simulink model "gm_HFMA_4B_1_5_9_13"  (R2026b)
settings: Solver=FixedStepDiscrete  StopTime=stopTime  FixedStep=1.953125e-06
PreLoadFcn:
  | load('a_luts.mat')
undefined symbols (not defined in the file or in its folder): Ts
libraries: simulink x202, simulink_need_slupdate x99, hdlsllib x91
(part 4 of 20)

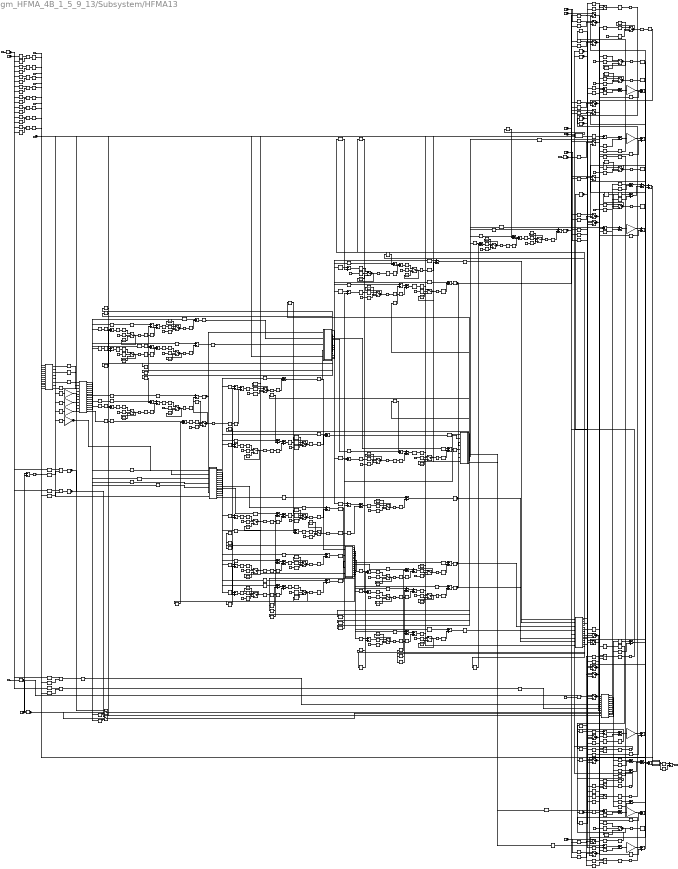
== system gm_HFMA_4B_1_5_9_13/Subsystem/HFMA13 ==
  Mic1 : Inport  OutDataTypeStr=fixdt(1, 20, 17)  PortDimensions=1  SampleTime=1.953125e-06
  Mic2 : Inport  Port=2  OutDataTypeStr=fixdt(1, 20, 17)  PortDimensions=1  SampleTime=1.953125e-06
  Mic3 : Inport  Port=3  OutDataTypeStr=fixdt(1, 20, 17)  PortDimensions=1  SampleTime=1.953125e-06
  Mic4 : Inport  Port=4  OutDataTypeStr=fixdt(1, 20, 17)  PortDimensions=1  SampleTime=1.953125e-06
  RESET : Inport  Port=5  OutDataTypeStr=boolean  PortDimensions=1  SampleTime=0.000125
  F0 Index : Inport  Port=6  OutDataTypeStr=fixdt(0, 18, 0)  PortDimensions=1  SampleTime=1.953125e-06
  IQ Counter : Inport  Port=7  OutDataTypeStr=uint8  PortDimensions=1  SampleTime=0.000125
  A Counter : Inport  Port=8  OutDataTypeStr=uint8  PortDimensions=1  SampleTime=0.000125
  sch_ctr_63 : Inport  Port=9  OutDataTypeStr=fixdt(0,6,0,'DataTypeOverride', 'Off')  PortDimensions=1  SampleTime=1.953125e-06
  Abs : Abs  SampleTime=1.953125e-06  OutDataTypeStr=fixdt(1, 18, 0)  SaturateOnIntegerOverflow=off
  Add : Sum  Inputs=+-  OutDataTypeStr=fixdt(1, 32, 29)  AccumDataTypeStr=fixdt(1, 33, 29)  SaturateOnIntegerOverflow=on  SampleTime=1.953125e-06
  Add1 : Sum  Inputs=+-  OutDataTypeStr=fixdt(1, 32, 29)  AccumDataTypeStr=fixdt(1, 33, 29)  SaturateOnIntegerOverflow=on  SampleTime=1.953125e-06
  Add{2..10} (9 alike) : Sum  OutDataTypeStr=fixdt(1, 32, 30)  AccumDataTypeStr=fixdt(1, 33, 30)  SaturateOnIntegerOverflow=on  SampleTime=1.953125e-06
  Add11 : Sum  OutDataTypeStr=fixdt(1, 32, 29)  AccumDataTypeStr=fixdt(1, 33, 29)  SaturateOnIntegerOverflow=on  SampleTime=1.953125e-06
  Add12 : Sum  OutDataTypeStr=fixdt(1, 32, 29)  AccumDataTypeStr=fixdt(1, 33, 29)  SaturateOnIntegerOverflow=on  SampleTime=1.953125e-06
  Add13 : Sum  Inputs=+-  OutDataTypeStr=fixdt(1, 32, 29)  AccumDataTypeStr=fixdt(1, 33, 29)  SaturateOnIntegerOverflow=on  SampleTime=1.953125e-06
  Add14 : Sum  OutDataTypeStr=fixdt(1, 32, 29)  AccumDataTypeStr=fixdt(1, 33, 29)  SaturateOnIntegerOverflow=on  SampleTime=1.953125e-06
  Add1_stage2 : Sum  OutDataTypeStr=fixdt(1, 34, 29)  AccumDataTypeStr=fixdt(1, 34, 29)  SaturateOnIntegerOverflow=on  SampleTime=1.953125e-06
  Add1_stage3 : Sum  OutDataTypeStr=fixdt(1, 32, 28)  AccumDataTypeStr=fixdt(1, 34, 29)  SaturateOnIntegerOverflow=on  SampleTime=1.953125e-06
  Add21 : Sum  OutDataTypeStr=fixdt(0, 40, 34)  AccumDataTypeStr=fixdt(0, 41, 34)  SaturateOnIntegerOverflow=on  SampleTime=1.953125e-06
  Add_stage2 : Sum  OutDataTypeStr=fixdt(1, 34, 29)  AccumDataTypeStr=fixdt(1, 34, 29)  SaturateOnIntegerOverflow=on  SampleTime=1.953125e-06
  Add_stage3 : Sum  OutDataTypeStr=fixdt(1, 32, 28)  AccumDataTypeStr=fixdt(1, 34, 29)  SaturateOnIntegerOverflow=on  SampleTime=1.953125e-06
  Compare : RelationalOperator  Operator===  OutDataTypeStr=boolean  SampleTime=1.953125e-06
  Constant : Constant  Value=90  OutDataTypeStr=fixdt(0, 18, 11)  SampleTime=1.953125e-06
  Constant1 : Constant  Value=180  OutDataTypeStr=uint8  SampleTime=1.953125e-06
  D1_{1..2,11..17,21..27} (16 alike) : RateTransition  OutPortSampleTimeOpt=Multiple of input port sample time  OutPortSampleTimeMultiple=64
  D1_1_absorbed{,1..7} (8 alike) : Delay  DelayLength=0
  D1_2_absorbed{,1..7} (8 alike) : Delay  DelayLength=0
  D2_{1..2,11..17,21..27} (16 alike) : RateTransition  OutPortSampleTimeOpt=Multiple of input port sample time  OutPortSampleTimeMultiple=64
  D2_1_absorbed{,1..7} (8 alike) : Delay  DelayLength=0
  D2_2_absorbed{,1..7} (8 alike) : Delay  DelayLength=0
  Delay1_bypass : Delay  DelayLength=1  InitialCondition=0  SampleTime=0.000125
  Delay1_bypass1 : RateTransition  OutPortSampleTimeOpt=Multiple of input port sample time  OutPortSampleTimeMultiple=64
  Delay1_lowered : RateTransition  OutPortSampleTimeOpt=Multiple of input port sample time  OutPortSampleTimeMultiple=64
  Delay1_lowered_absorbed : Delay  DelayLength=0
  Delay2_bypass : Delay  DelayLength=1  InitialCondition=0  SampleTime=0.000125
  Delay2_bypass1 : RateTransition  OutPortSampleTimeOpt=Multiple of input port sample time  OutPortSampleTimeMultiple=64
  Delay2_lowered : RateTransition  OutPortSampleTimeOpt=Multiple of input port sample time  OutPortSampleTimeMultiple=64
  Delay2_lowered_absorbed : Delay  DelayLength=0
  Delay3_bypass : Delay  DelayLength=1  InitialCondition=0  SampleTime=0.000125
  Delay3_bypass1 : RateTransition  OutPortSampleTimeOpt=Multiple of input port sample time  OutPortSampleTimeMultiple=64
  Delay3_lowered : RateTransition  OutPortSampleTimeOpt=Multiple of input port sample time  OutPortSampleTimeMultiple=64
  Delay3_lowered_absorbed : Delay  DelayLength=0
  Delay4_bypass : Delay  DelayLength=1  InitialCondition=0  SampleTime=0.000125
  Delay4_bypass1 : RateTransition  OutPortSampleTimeOpt=Multiple of input port sample time  OutPortSampleTimeMultiple=64
  Delay4_lowered : RateTransition  OutPortSampleTimeOpt=Multiple of input port sample time  OutPortSampleTimeMultiple=64
  Delay4_lowered_absorbed : Delay  DelayLength=0
  Delay5_bypass : Delay  DelayLength=1  InitialCondition=0  SampleTime=0.000125
  Delay5_bypass1 : RateTransition  OutPortSampleTimeOpt=Multiple of input port sample time  OutPortSampleTimeMultiple=64
  Delay5_lowered : RateTransition  OutPortSampleTimeOpt=Multiple of input port sample time  OutPortSampleTimeMultiple=64
  Delay5_lowered_absorbed : Delay  DelayLength=0
  Delay_Switch{,1..5} (6 alike) : Switch  Criteria=u2 ~= 0  OutDataTypeStr=fixdt(1, 32, 30)  SampleTime=1.953125e-06  SaturateOnIntegerOverflow=off  InputSameDT=off
  Delay_bypass : Delay  DelayLength=1  InitialCondition=0  SampleTime=0.000125
  Delay_bypass1 : RateTransition  OutPortSampleTimeOpt=Multiple of input port sample time  OutPortSampleTimeMultiple=64
  Delay_lowered{,1..6} (7 alike) : RateTransition  OutPortSampleTimeOpt=Multiple of input port sample time  OutPortSampleTimeMultiple=64
  Delay_lowered_absorbed{,1..6} (7 alike) : Delay  DelayLength=0
  Delay_toDelbypassMux{,1..5} (6 alike) : Switch  Criteria=u2 ~= 0  OutDataTypeStr=fixdt(1, 32, 30)  SampleTime=0.000125  SaturateOnIntegerOverflow=off  InputSameDT=off
  Direct Lookup Table (n-D) : LookupNDDirect  Table="reshape(fi([0.999969482421875;0.999969482421875;0.999969482421875;0.999969482421875;0.999969482421875;0.999969482421875;0.999969482421875;0.999969482421875;0.999969482421875;0.999969482421875;0.999969482421875;0.999969482421875;0.999969482421875;0.999969482421875;0.999969482421875;0.999969482421875;0.999969482421875;0.999969482421875;0.99993896484375;0.999908447265625;0.9998779296875;0.99981689453125;0.999755859375;0.99969482421875;0.9996337890625;0.99957275390625;0.999481201171875;0.9993896484375;0.999298095703125;0.999176025390625;0.99908447265625;0.99896240234375;0.99993896484375;0.9998779296875;0.999755859375;0.9996337890625;0.999481201171875;0.999298095703125;0.99908447265625;0.99884033203125;0.998565673828125;0.998260498046875;0.9979248046875;0.99755859375;0.997161865234375;0.99676513671875;0.996307373046875;0.995849609375;0.9998779296875;0.99969482421875;0.999481201171875;0.999176025390625;0.99884033203125;0.9984130859375;0.9979248046875;0.99737548828125;0.99676513671875;0.99609375;0.995330810546875;0.994537353515625;0.99365234375;0.992706298828125;0.99169921875;0.990631103515625;0.999755859375;0.999481201171875;0.99908447265625;0.998565673828125;0.9979248046875;0.9971923828125;0.996307373046875;0.995330810546875;0.994232177734375;0.9930419921875;0.991729736328125;0.99029541015625;0.988739013671875;0.987060546875;0.98529052734375;0.9833984375;0.9996337890625;0.999176025390625;0.998565673828125;0.99774169921875;0.99676513671875;0.99560546875;0.9942626953125;0.99273681640625;0.99102783203125;0.9891357421875;0.987091064453125;0.984832763671875;0.982421875;0.979827880859375;0.977081298828125;0.97412109375;0.999481201171875;0.99884033203125;0.9979248046875;0.99676513671875;0.995361328125;0.993682861328125;0.991729736328125;0.989532470703125;0.987091064453125;0.984375;0.9814453125;0.97821044921875;0.974761962890625;0.971038818359375;0.967071533203125;0.962860107421875;0.999298095703125;0.9984130859375;0.9971923828125;0.99560546875;0.993682861328125;0.99139404296875;0.98876953125;0.98577880859375;0.98248291015625;0.978790283203125;0.97479248046875;0.970428466796875;0.965728759765625;0.960693359375;0.955322265625;0.949615478515625;0.99908447265625;0.9979248046875;0.996337890625;0.9942626953125;0.99176025390625;0.988800048828125;0.9853515625;0.981475830078125;0.977142333984375;0.972381591796875;0.9671630859375;0.96148681640625;0.95538330078125;0.9488525390625;0.941864013671875;0.9344482421875;0.99884033203125;0.997406005859375;0.995361328125;0.992767333984375;0.989593505859375;0.98583984375;0.98150634765625;0.97662353515625;0.971160888671875;0.96514892578125;0.95855712890625;0.951446533203125;0.943756103515625;0.935516357421875;0.9267578125;0.917449951171875;0.998565673828125;0.996795654296875;0.994293212890625;0.9910888671875;0.9871826171875;0.9825439453125;0.97723388671875;0.971221923828125;0.964508056640625;0.957122802734375;0.94903564453125;0.940277099609375;0.93084716796875;0.920745849609375;0.910003662109375;0.898590087890625;0.998291015625;0.996124267578125;0.99310302734375;0.9892578125;0.984527587890625;0.97894287109375;0.9725341796875;0.965301513671875;0.95721435546875;0.94830322265625;0.938568115234375;0.92803955078125;0.916717529296875;0.904571533203125;0.89166259765625;0.87799072265625;0.997955322265625;0.995391845703125;0.9918212890625;0.98724365234375;0.98162841796875;0.97503662109375;0.967437744140625;0.958831787109375;0.949249267578125;0.938720703125;0.927215576171875;0.914764404296875;0.9013671875;0.887054443359375;0.871826171875;0.855712890625;0.99761962890625;0.994598388671875;0.99041748046875;0.98504638671875;0.978515625;0.970794677734375;0.9619140625;0.951873779296875;0.940673828125;0.928375244140625;0.91497802734375;0.90045166015625;0.884857177734375;0.86822509765625;0.85052490234375;0.831817626953125;0.997222900390625;0.9937744140625;0.988922119140625;0.98272705078125;0.97515869140625;0.96624755859375;0.95599365234375;0.94439697265625;0.9315185546875;0.917327880859375;0.901885986328125;0.885162353515625 ...(+21044 chars)), [16  91])"  SampleTime=1.953125e-06  TableDataTypeStr=fixdt(1,18,16)
  Direct Lookup Table (n-D)1 : LookupNDDirect  Table="reshape(fi([0;0;0;0;0;0;0;0;0;0;0;0;0;0;0;0;-0.00537109375;-0.008056640625;-0.0107421875;-0.013427734375;-0.01611328125;-0.018798828125;-0.021484375;-0.024169921875;-0.02685546875;-0.029541015625;-0.0322265625;-0.034912109375;-0.03759765625;-0.040283203125;-0.04296875;-0.045623779296875;-0.0107421875;-0.01611328125;-0.021484375;-0.02685546875;-0.0322265625;-0.037567138671875;-0.042938232421875;-0.048309326171875;-0.053680419921875;-0.059051513671875;-0.06439208984375;-0.06976318359375;-0.075103759765625;-0.080474853515625;-0.0858154296875;-0.091156005859375;-0.01611328125;-0.024169921875;-0.032196044921875;-0.040252685546875;-0.048309326171875;-0.05633544921875;-0.06439208984375;-0.072418212890625;-0.0804443359375;-0.088470458984375;-0.09649658203125;-0.1044921875;-0.112518310546875;-0.120513916015625;-0.12847900390625;-0.136474609375;-0.021453857421875;-0.032196044921875;-0.04290771484375;-0.05364990234375;-0.064361572265625;-0.0750732421875;-0.08575439453125;-0.096466064453125;-0.10711669921875;-0.1177978515625;-0.128448486328125;-0.13909912109375;-0.14971923828125;-0.160308837890625;-0.1708984375;-0.18145751953125;-0.026824951171875;-0.04022216796875;-0.053619384765625;-0.0670166015625;-0.08038330078125;-0.09375;-0.107086181640625;-0.120391845703125;-0.133697509765625;-0.14697265625;-0.160247802734375;-0.1734619140625;-0.1866455078125;-0.199798583984375;-0.212921142578125;-0.22601318359375;-0.03216552734375;-0.048248291015625;-0.064300537109375;-0.080322265625;-0.096343994140625;-0.11236572265625;-0.128326416015625;-0.144256591796875;-0.16015625;-0.175994873046875;-0.191802978515625;-0.20758056640625;-0.2232666015625;-0.238922119140625;-0.2545166015625;-0.270050048828125;-0.037506103515625;-0.05621337890625;-0.074951171875;-0.0936279296875;-0.112274169921875;-0.130889892578125;-0.149444580078125;-0.16796875;-0.186431884765625;-0.204803466796875;-0.22314453125;-0.241363525390625;-0.259521484375;-0.277587890625;-0.295562744140625;-0.31341552734375;-0.042816162109375;-0.064208984375;-0.085540771484375;-0.10687255859375;-0.128143310546875;-0.14935302734375;-0.17047119140625;-0.191558837890625;-0.2125244140625;-0.2333984375;-0.254150390625;-0.274810791015625;-0.29534912109375;-0.31573486328125;-0.335968017578125;-0.3560791015625;-0.048126220703125;-0.0721435546875;-0.09613037109375;-0.12005615234375;-0.1439208984375;-0.167694091796875;-0.191375732421875;-0.214935302734375;-0.2384033203125;-0.261688232421875;-0.28485107421875;-0.307830810546875;-0.330657958984375;-0.353271484375;-0.375701904296875;-0.39788818359375;-0.05340576171875;-0.080078125;-0.106689453125;-0.133209228515625;-0.159637451171875;-0.185943603515625;-0.212127685546875;-0.2381591796875;-0.2640380859375;-0.289703369140625;-0.315185546875;-0.340423583984375;-0.36541748046875;-0.390167236328125;-0.41461181640625;-0.43878173828125;-0.058685302734375;-0.087982177734375;-0.1171875;-0.146270751953125;-0.175262451171875;-0.204071044921875;-0.23272705078125;-0.26116943359375;-0.289398193359375;-0.3173828125;-0.3450927734375;-0.37249755859375;-0.399566650390625;-0.426300048828125;-0.452667236328125;-0.478668212890625;-0.063934326171875;-0.0958251953125;-0.12762451171875;-0.159271240234375;-0.190765380859375;-0.222076416015625;-0.253143310546875;-0.283966064453125;-0.314483642578125;-0.344696044921875;-0.374542236328125;-0.404022216796875;-0.433074951171875;-0.461669921875;-0.48980712890625;-0.5174560546875;-0.069183349609375;-0.103668212890625;-0.13800048828125;-0.172210693359375;-0.206207275390625;-0.23992919921875;-0.27337646484375;-0.3065185546875;-0.339263916015625;-0.371612548828125;-0.403533935546875;-0.4349365234375;-0.465850830078125;-0.496185302734375;-0.52593994140625;-0.5550537109375;-0.074371337890625;-0.1114501953125;-0.148345947265625;-0.18505859375;-0.22149658203125;-0.25762939453125;-0.293426513671875;-0.32879638671875;-0.36370849609375;-0.39813232421875;-0.4320068359375;-0.46527099609375;-0.497894287109375;-0.529815673828125;-0.561004638671875;-0.5914306640625 ...(+21853 chars)), [16  91])"  SampleTime=1.953125e-06  TableDataTypeStr=fixdt(1,18,16)
  Direct Lookup Table (n-D)2 : LookupNDDirect  Table="reshape(fi([0.999969482421875;0.999969482421875;0.999969482421875;0.999969482421875;0.999969482421875;0.999969482421875;0.999969482421875;0.999969482421875;0.999969482421875;0.999969482421875;0.999969482421875;0.999969482421875;0.999969482421875;0.999969482421875;0.999969482421875;0.999969482421875;0.99993896484375;0.9998779296875;0.999755859375;0.9996337890625;0.999481201171875;0.999298095703125;0.99908447265625;0.99884033203125;0.998565673828125;0.998260498046875;0.9979248046875;0.99755859375;0.997161865234375;0.99676513671875;0.996307373046875;0.995849609375;0.999755859375;0.999481201171875;0.99908447265625;0.998565673828125;0.9979248046875;0.997161865234375;0.996307373046875;0.995330810546875;0.994232177734375;0.9930419921875;0.99169921875;0.990264892578125;0.98870849609375;0.987060546875;0.985260009765625;0.983367919921875;0.999481201171875;0.99884033203125;0.9979248046875;0.99676513671875;0.995330810546875;0.99365234375;0.99169921875;0.989501953125;0.987060546875;0.984344482421875;0.98138427734375;0.9781494140625;0.97467041015625;0.970947265625;0.96697998046875;0.962738037109375;0.99908447265625;0.9979248046875;0.996307373046875;0.994232177734375;0.991729736328125;0.988739013671875;0.98529052734375;0.98138427734375;0.97705078125;0.972259521484375;0.967010498046875;0.9613037109375;0.955169677734375;0.9486083984375;0.94158935546875;0.93414306640625;0.998565673828125;0.99676513671875;0.9942626953125;0.99102783203125;0.987091064453125;0.982421875;0.977081298828125;0.97100830078125;0.9642333984375;0.956787109375;0.948638916015625;0.9398193359375;0.930328369140625;0.920166015625;0.909332275390625;0.8978271484375;0.9979248046875;0.995361328125;0.991729736328125;0.987091064453125;0.9814453125;0.974761962890625;0.967071533203125;0.9583740234375;0.948699951171875;0.93804931640625;0.926422119140625;0.913818359375;0.900299072265625;0.885833740234375;0.870452880859375;0.854156494140625;0.9971923828125;0.993682861328125;0.98876953125;0.98248291015625;0.97479248046875;0.965728759765625;0.955322265625;0.943572998046875;0.93048095703125;0.916107177734375;0.900421142578125;0.88348388671875;0.86529541015625;0.84588623046875;0.825286865234375;0.80352783203125;0.996337890625;0.99176025390625;0.9853515625;0.977142333984375;0.9671630859375;0.95538330078125;0.941864013671875;0.9266357421875;0.90966796875;0.89105224609375;0.87078857421875;0.848968505859375;0.8255615234375;0.800628662109375;0.77423095703125;0.746429443359375;0.995361328125;0.989593505859375;0.98150634765625;0.971160888671875;0.95855712890625;0.943756103515625;0.9267578125;0.9075927734375;0.886322021484375;0.863037109375;0.83770751953125;0.810455322265625;0.781341552734375;0.750396728515625;0.71771240234375;0.683380126953125;0.994293212890625;0.9871826171875;0.97723388671875;0.964508056640625;0.94903564453125;0.93084716796875;0.910003662109375;0.886566162109375;0.860565185546875;0.8321533203125;0.80133056640625;0.768218994140625;0.732940673828125;0.695556640625;0.65618896484375;0.614959716796875;0.99310302734375;0.984527587890625;0.9725341796875;0.95721435546875;0.938568115234375;0.916717529296875;0.89166259765625;0.863555908203125;0.832489013671875;0.798553466796875;0.7618408203125;0.722503662109375;0.680694580078125;0.63653564453125;0.59014892578125;0.541778564453125;0.9918212890625;0.98162841796875;0.967437744140625;0.949249267578125;0.927215576171875;0.9013671875;0.871826171875;0.838714599609375;0.80218505859375;0.762359619140625;0.71942138671875;0.673553466796875;0.624908447265625;0.573699951171875;0.520172119140625;0.464508056640625;0.99041748046875;0.978515625;0.9619140625;0.940673828125;0.91497802734375;0.884857177734375;0.85052490234375;0.812103271484375;0.769805908203125;0.723785400390625;0.67431640625;0.62164306640625;0.565948486328125;0.507568359375;0.44677734375;0.383819580078125;0.988922119140625;0.97515869140625;0.95599365234375;0.9315185546875;0.901885986328125;0.86724853515625;0.82781982421875;0.783782958984375;0.73541259765625;0.6829833984375;0.62677001953125 ...(+21447 chars)), [16  91])"  SampleTime=1.953125e-06  TableDataTypeStr=fixdt(1,18,16)
  Direct Lookup Table (n-D)3 : LookupNDDirect  Table="reshape(fi([0;0;0;0;0;0;0;0;0;0;0;0;0;0;0;0;-0.0107421875;-0.01611328125;-0.021484375;-0.02685546875;-0.0322265625;-0.03759765625;-0.04296875;-0.048309326171875;-0.053680419921875;-0.059051513671875;-0.06439208984375;-0.06976318359375;-0.07513427734375;-0.080474853515625;-0.0858154296875;-0.0911865234375;-0.021484375;-0.0322265625;-0.042938232421875;-0.053680419921875;-0.06439208984375;-0.075103759765625;-0.0858154296875;-0.09649658203125;-0.107208251953125;-0.11785888671875;-0.1285400390625;-0.13916015625;-0.149810791015625;-0.160400390625;-0.170989990234375;-0.18157958984375;-0.032196044921875;-0.048309326171875;-0.06439208984375;-0.0804443359375;-0.09649658203125;-0.112518310546875;-0.12847900390625;-0.144439697265625;-0.160369873046875;-0.176239013671875;-0.19207763671875;-0.207855224609375;-0.22357177734375;-0.2392578125;-0.254852294921875;-0.2703857421875;-0.04290771484375;-0.064361572265625;-0.08575439453125;-0.10711669921875;-0.128448486328125;-0.14971923828125;-0.1708984375;-0.1920166015625;-0.213043212890625;-0.23394775390625;-0.2547607421875;-0.275482177734375;-0.296051025390625;-0.31646728515625;-0.336761474609375;-0.356903076171875;-0.053619384765625;-0.08038330078125;-0.107086181640625;-0.133697509765625;-0.160247802734375;-0.1866455078125;-0.212921142578125;-0.23907470703125;-0.2650146484375;-0.290771484375;-0.31634521484375;-0.3416748046875;-0.36676025390625;-0.391571044921875;-0.416107177734375;-0.440338134765625;-0.064300537109375;-0.096343994140625;-0.128326416015625;-0.16015625;-0.191802978515625;-0.2232666015625;-0.2545166015625;-0.285491943359375;-0.316162109375;-0.346527099609375;-0.376495361328125;-0.406097412109375;-0.435302734375;-0.464019775390625;-0.492279052734375;-0.52001953125;-0.074951171875;-0.112274169921875;-0.149444580078125;-0.186431884765625;-0.22314453125;-0.259521484375;-0.295562744140625;-0.3311767578125;-0.3663330078125;-0.40093994140625;-0.435028076171875;-0.468475341796875;-0.50128173828125;-0.533355712890625;-0.564697265625;-0.595245361328125;-0.085540771484375;-0.128143310546875;-0.17047119140625;-0.2125244140625;-0.254150390625;-0.29534912109375;-0.335968017578125;-0.376007080078125;-0.415313720703125;-0.453887939453125;-0.49163818359375;-0.528472900390625;-0.5643310546875;-0.599151611328125;-0.632904052734375;-0.66546630859375;-0.09613037109375;-0.1439208984375;-0.191375732421875;-0.2384033203125;-0.28485107421875;-0.330657958984375;-0.375701904296875;-0.41986083984375;-0.463043212890625;-0.505157470703125;-0.546112060546875;-0.585784912109375;-0.624114990234375;-0.660980224609375;-0.696319580078125;-0.730072021484375;-0.106689453125;-0.159637451171875;-0.212127685546875;-0.2640380859375;-0.315185546875;-0.36541748046875;-0.41461181640625;-0.462615966796875;-0.50933837890625;-0.5545654296875;-0.59820556640625;-0.640167236328125;-0.6802978515625;-0.718475341796875;-0.754608154296875;-0.78857421875;-0.1171875;-0.175262451171875;-0.23272705078125;-0.289398193359375;-0.3450927734375;-0.399566650390625;-0.452667236328125;-0.504241943359375;-0.554046630859375;-0.6019287109375;-0.64776611328125;-0.691375732421875;-0.732574462890625;-0.771270751953125;-0.807281494140625;-0.84051513671875;-0.12762451171875;-0.190765380859375;-0.253143310546875;-0.314483642578125;-0.374542236328125;-0.433074951171875;-0.48980712890625;-0.5445556640625;-0.597076416015625;-0.64715576171875;-0.694549560546875;-0.7391357421875;-0.78070068359375;-0.819061279296875;-0.85406494140625;-0.885589599609375;-0.13800048828125;-0.206207275390625;-0.27337646484375;-0.339263916015625;-0.403533935546875;-0.465850830078125;-0.52593994140625;-0.583526611328125;-0.6383056640625;-0.69000244140625;-0.738433837890625;-0.783294677734375;-0.824432373046875;-0.861602783203125;-0.8946533203125;-0.92340087890625;-0.148345947265625;-0.22149658203125;-0.293426513671875;-0.36370849609375;-0.4320068359375;-0.497894287109375;-0.561004638671875;-0.62103271484375;-0.6776123046875;-0.730438232421875;-0.779205322265625;-0.82366943359375 ...(+21735 chars)), [16  91])"  SampleTime=1.953125e-06  TableDataTypeStr=fixdt(1,18,16)
  Gain{,1..5} (6 alike) : Gain  Gain="fi(0,1,32,40,\"hex\",\"40000000\")"  ParamDataTypeStr=fixdt(1, 32, 40)  OutDataTypeStr=fixdt(1, 32, 30)  SaturateOnIntegerOverflow=on  SampleTime=1.953125e-06
  Gain{11..14} (4 alike) : Gain  Gain="fi(0,0,18,16,\"hex\",\"20000\")"  ParamDataTypeStr=fixdt(0, 18, 16)  OutDataTypeStr=fixdt(1, 18, 14)  SaturateOnIntegerOverflow=on  SampleTime=1.953125e-06
  Gain1_out_dtc : DataTypeConversion  OutDataTypeStr=fixdt(0, 18, 17)  SampleTime=1.953125e-06  RndMeth=Floor
  Gain_out_dtc : DataTypeConversion  OutDataTypeStr=fixdt(1, 18, 16)  SampleTime=1.953125e-06  RndMeth=Floor
  Gain_out_dtc{1..4} (4 alike) : DataTypeConversion  OutDataTypeStr=fixdt(1, 18, 14)  SampleTime=1.953125e-06  RndMeth=Floor
  IdxConv{,2..10,14..15,21..24} (16 alike) : DataTypeConversion  OutDataTypeStr=uint8  SampleTime=1.953125e-06  RndMeth=Floor
  IdxConv{1,11..13,31..34} (8 alike) : DataTypeConversion  OutDataTypeStr=fixdt('uint8')
  Initial_Val{,1..5} (6 alike) : Constant  Value=0  OutDataTypeStr=fixdt(1, 32, 30)  SampleTime=1.953125e-06
  Minus{,1..5} (6 alike) : Sum  Inputs=+-  OutDataTypeStr=fixdt(1, 32, 30)  AccumDataTypeStr=fixdt(1, 33, 30)  SaturateOnIntegerOverflow=on  SampleTime=1.953125e-06
  PipelineRegister{,1..11} (12 alike) : Delay  DelayLength=1  InitialCondition=0  SampleTime=1.953125e-06
  Product1_out_dtc : DataTypeConversion  OutDataTypeStr=fixdt(1, 32, 29)  SampleTime=1.953125e-06  RndMeth=Floor
  Product1_out_dtc1 : DataTypeConversion  OutDataTypeStr=fixdt(1, 32, 29)  SampleTime=1.953125e-06  RndMeth=Floor
  Product1_out_dtc{4,6..8,10..11} (6 alike) : DataTypeConversion  OutDataTypeStr=fixdt(1, 32, 30)  SampleTime=1.953125e-06  RndMeth=Floor
  Product1_out_dtc{3,5,9,12} (4 alike) : DataTypeConversion  OutDataTypeStr=fixdt(1, 18, 15)  SampleTime=1.953125e-06  RndMeth=Floor
  Product1_out_dtc13 : DataTypeConversion  OutDataTypeStr=fixdt(0, 40, 34)  SampleTime=1.953125e-06  RndMeth=Floor
  Product1_out_dtc2 : DataTypeConversion  OutDataTypeStr=fixdt(1, 32, 29)  SampleTime=1.953125e-06  RndMeth=Floor
  Product2_out_dtc : DataTypeConversion  OutDataTypeStr=fixdt(1, 32, 29)  SampleTime=1.953125e-06  RndMeth=Floor
  Product2_out_dtc1 : DataTypeConversion  OutDataTypeStr=fixdt(1, 32, 29)  SampleTime=1.953125e-06  RndMeth=Floor
  Product2_out_dtc2 : DataTypeConversion  OutDataTypeStr=fixdt(1, 32, 29)  SampleTime=1.953125e-06  RndMeth=Floor
  Product3_out_dtc : DataTypeConversion  OutDataTypeStr=fixdt(1, 32, 29)  SampleTime=1.953125e-06  RndMeth=Floor
  Product3_out_dtc1 : DataTypeConversion  OutDataTypeStr=fixdt(1, 32, 29)  SampleTime=1.953125e-06  RndMeth=Floor
  Product3_out_dtc2 : DataTypeConversion  OutDataTypeStr=fixdt(1, 32, 29)  SampleTime=1.953125e-06  RndMeth=Floor
  Product_out_dtc : DataTypeConversion  OutDataTypeStr=fixdt(1, 32, 29)  SampleTime=1.953125e-06  RndMeth=Floor
  Product_out_dtc1 : DataTypeConversion  OutDataTypeStr=fixdt(1, 32, 29)  SampleTime=1.953125e-06  RndMeth=Floor
  Product_out_dtc{3..4,6,8,10..11} (6 alike) : DataTypeConversion  OutDataTypeStr=fixdt(1, 32, 30)  SampleTime=1.953125e-06  RndMeth=Floor
  Product_out_dtc12 : DataTypeConversion  OutDataTypeStr=fixdt(1, 32, 29)  SampleTime=1.953125e-06  RndMeth=Floor
  Product_out_dtc13 : DataTypeConversion  OutDataTypeStr=fixdt(0, 40, 34)  SampleTime=1.953125e-06  RndMeth=Floor
  Product_out_dtc{2,5,7,9} (4 alike) : DataTypeConversion  OutDataTypeStr=fixdt(1, 18, 15)  SampleTime=1.953125e-06  RndMeth=Floor
  Q_{1..2,11..17,21..27} (16 alike) : DataTypeConversion  OutDataTypeStr=fixdt(1, 18, 16)  SampleTime=1.953125e-06  RndMeth=Floor
  Relational Operator : RelationalOperator  OutDataTypeStr=boolean  SampleTime=1.953125e-06  InputSameDT=off
  S0_{1..2,11..17,21..27} (16 alike) : Sum  OutDataTypeStr=fixdt(1, 40, 30)  AccumDataTypeStr=fixdt(1, 41, 30)  SaturateOnIntegerOverflow=on  SampleTime=1.953125e-06
  S1_1_out1bypassMux{,1..7} (8 alike) : Switch  Criteria=u2 ~= 0  OutDataTypeStr=fixdt(1, 40, 30)  SampleTime=0.000125  SaturateOnIntegerOverflow=off  InputSameDT=off
  S1_1_stage{2,21..27} (8 alike) : Sum  OutDataTypeStr=fixdt(1, 42, 30)  AccumDataTypeStr=fixdt(1, 42, 30)  SaturateOnIntegerOverflow=on  SampleTime=1.953125e-06
  S1_1_stage{3,31..37} (8 alike) : Sum  OutDataTypeStr=fixdt(1, 40, 30)  AccumDataTypeStr=fixdt(1, 42, 30)  SaturateOnIntegerOverflow=on  SampleTime=1.953125e-06
  S1_2_out1bypassMux{,1..7} (8 alike) : Switch  Criteria=u2 ~= 0  OutDataTypeStr=fixdt(1, 40, 30)  SampleTime=0.000125  SaturateOnIntegerOverflow=off  InputSameDT=off
  S1_2_stage{2,21..27} (8 alike) : Sum  OutDataTypeStr=fixdt(1, 42, 30)  AccumDataTypeStr=fixdt(1, 42, 30)  SaturateOnIntegerOverflow=on  SampleTime=1.953125e-06
  S1_2_stage{3,31..37} (8 alike) : Sum  OutDataTypeStr=fixdt(1, 40, 30)  AccumDataTypeStr=fixdt(1, 42, 30)  SaturateOnIntegerOverflow=on  SampleTime=1.953125e-06
  S2_{1..2,11..17,21..27} (16 alike) : Sum  OutDataTypeStr=fixdt(1, 40, 30)  AccumDataTypeStr=fixdt(1, 41, 30)  SaturateOnIntegerOverflow=on  SampleTime=1.953125e-06
  S2_1_out1bypassMux{,1..7} (8 alike) : Switch  Criteria=u2 ~= 0  OutDataTypeStr=fixdt(1, 40, 30)  SampleTime=0.000125  SaturateOnIntegerOverflow=off  InputSameDT=off
  S2_2_out1bypassMux{,1..7} (8 alike) : Switch  Criteria=u2 ~= 0  OutDataTypeStr=fixdt(1, 40, 30)  SampleTime=0.000125  SaturateOnIntegerOverflow=off  InputSameDT=off
  Subtract : Sum  Inputs=+-  OutDataTypeStr=fixdt(1, 18, 0)  AccumDataTypeStr=fixdt(1, 20, 11)  SaturateOnIntegerOverflow=on  SampleTime=1.953125e-06
  Subtract1 : Sum  Inputs=+-  OutDataTypeStr=fixdt(1, 32, 30)  AccumDataTypeStr=fixdt(1, 33, 30)  SaturateOnIntegerOverflow=on  SampleTime=1.953125e-06
  Subtract2 : Sum  Inputs=+-  OutDataTypeStr=fixdt(1, 32, 30)  AccumDataTypeStr=fixdt(1, 33, 30)  SaturateOnIntegerOverflow=on  SampleTime=1.953125e-06
  Subtract3 : Sum  Inputs=+-  OutDataTypeStr=fixdt(1, 32, 30)  AccumDataTypeStr=fixdt(1, 33, 30)  SaturateOnIntegerOverflow=on  SampleTime=1.953125e-06
  Switch : Switch  Criteria=u2 ~= 0  Threshold="fi(0,0,1,0,\"hex\",\"0\")"  OutDataTypeStr=fixdt(1, 18, 16)  SampleTime=1.953125e-06  SaturateOnIntegerOverflow=off  InputSameDT=off
  Switch1 : Switch  Criteria=u2 ~= 0  Threshold="fi(0,0,1,0,\"hex\",\"0\")"  OutDataTypeStr=fixdt(1, 18, 16)  SampleTime=1.953125e-06  SaturateOnIntegerOverflow=off  InputSameDT=off
  b0_1_out_dtc{,1..7} (8 alike) : DataTypeConversion  OutDataTypeStr=fixdt(1, 40, 30)  SampleTime=1.953125e-06  RndMeth=Floor
  b0_2_out_dtc{,1..7} (8 alike) : DataTypeConversion  OutDataTypeStr=fixdt(1, 40, 30)  SampleTime=1.953125e-06  RndMeth=Floor
  b1_1_out_dtc{,1..7} (8 alike) : DataTypeConversion  OutDataTypeStr=fixdt(1, 40, 30)  SampleTime=1.953125e-06  RndMeth=Floor
  b1_2_out_dtc{,1..7} (8 alike) : DataTypeConversion  OutDataTypeStr=fixdt(1, 40, 30)  SampleTime=1.953125e-06  RndMeth=Floor
  b2_1_out_dtc{,1..7} (8 alike) : DataTypeConversion  OutDataTypeStr=fixdt(1, 40, 30)  SampleTime=1.953125e-06  RndMeth=Floor
  b2_2_out_dtc{,1..7} (8 alike) : DataTypeConversion  OutDataTypeStr=fixdt(1, 40, 30)  SampleTime=1.953125e-06  RndMeth=Floor
  bypass_out{,1..5} (6 alike) : Switch  Criteria=u2 ~= 0  OutDataTypeStr=fixdt(1, 32, 30)  SampleTime=1.953125e-06  SaturateOnIntegerOverflow=off  InputSameDT=off
  cosLUT{,1..3} (4 alike) : LookupNDDirect  Table="reshape([1;1;1;1;1;1;1;1;1;1;1;1;1;1;1;1;0.95105651629515353;0.8910065241883679;0.80901699437494745;0.70710678118654757;0.58778525229247314;0.45399049973954686;0.30901699437494745;0.15643446504023092;6.123233995736766e-17;-0.15643446504023081;-0.30901699437494734;-0.45399049973954675;-0.58778525229247303;-0.70710678118654746;-0.80901699437494734;-0.89100652418836779;0.80901699437494745;0.58778525229247314;0.30901699437494745;6.123233995736766e-17;-0.30901699437494734;-0.58778525229247303;-0.80901699437494734;-0.95105651629515353;-1;-0.95105651629515364;-0.80901699437494745;-0.58778525229247325;-0.30901699437494756;-1.8369701987210297e-16;0.30901699437494723;0.58778525229247292;0.58778525229247314;0.15643446504023092;-0.30901699437494734;-0.70710678118654746;-0.95105651629515353;-0.98768834059513777;-0.80901699437494745;-0.45399049973954692;-1.8369701987210297e-16;0.45399049973954664;0.80901699437494734;0.98768834059513755;0.95105651629515398;0.70710678118654835;0.30901699437494773;-0.15643446504022968;0.30901699437494745;-0.30901699437494734;-0.80901699437494734;-1;-0.80901699437494745;-0.30901699437494756;0.30901699437494723;0.80901699437494734;1;0.80901699437494756;0.30901699437494773;-0.30901699437494712;-0.80901699437494723;-1;-0.80901699437494767;-0.30901699437494784;-1.6081226496766366e-16;-0.70710678118654746;-1;-0.70710678118654791;-1.8369701987210297e-16;0.70710678118654735;1;0.70710678118654835;1.1943401194869635e-15;-0.70710678118654791;-1;-0.70710678118654846;-4.2862637970157361e-16;0.70710678118654779;1;0.70710678118654857;-0.30901699437494734;-0.95105651629515353;-0.80901699437494745;-1.8369701987210297e-16;0.80901699437494734;0.95105651629515398;0.30901699437494773;-0.58778525229247292;-1;-0.58778525229247347;0.30901699437494701;0.95105651629515287;0.80901699437494878;2.3274478990165594e-15;-0.80901699437494712;-0.95105651629515431;-0.58778525229247336;-0.98768834059513777;-0.30901699437494673;0.70710678118654735;0.95105651629515364;0.15643446504023203;-0.80901699437494823;-0.89100652418836768;-4.2862637970157361e-16;0.89100652418836801;0.80901699437494778;-0.15643446504022945;-0.95105651629515287;-0.70710678118654735;0.30901699437495017;0.98768834059513744;-0.80901699437494734;-0.80901699437494745;0.30901699437494723;1;0.30901699437494773;-0.80901699437494723;-0.80901699437494767;0.30901699437494701;1;0.30901699437494795;-0.80901699437494712;-0.80901699437494778;0.30901699437494679;1;0.30901699437494817;-0.8090169943749469;-0.95105651629515353;-0.45399049973954692;0.80901699437494734;0.70710678118654835;-0.58778525229247292;-0.89100652418836845;0.30901699437494701;0.98768834059513799;2.3274478990165594e-15;-0.98768834059513777;-0.30901699437494806;0.89100652418836634;0.58778525229247514;-0.70710678118654635;-0.8090169943749479;0.45399049973954675;-1;-1.8369701987210297e-16;1;1.1943401194869635e-15;-1;-4.2862637970157361e-16;1;2.3274478990165594e-15;-1;1.1028010998692062e-15;1;2.5723772588460301e-15;-1;8.5787174003973557e-16;1;2.8173066186755008e-15;-0.95105651629515364;0.45399049973954581;0.80901699437494756;-0.70710678118654668;-0.58778525229247491;0.89100652418836723;0.30901699437494795;-0.98768834059513777;-2.4499125789312946e-15;0.98768834059513766;-0.30901699437494329;-0.89100652418836868;0.58778525229247092;0.70710678118654757;-0.80901699437494679;-0.45399049973955174;-0.80901699437494745;0.80901699437494734;0.30901699437494773;-1;0.30901699437494701;0.80901699437494878;-0.80901699437494712;-0.30901699437494806;1;-0.30901699437494667;-0.8090169943749479;0.80901699437494479;0.30901699437495178;-1;0.30901699437494629;0.80901699437495023;-0.58778525229247325;0.98768834059513766;-0.30901699437494712;-0.70710678118654846;0.95105651629515342;-0.15643446504022945;-0.80901699437494778;0.8910065241883679;2.5723772588460301e-15;-0.89100652418836701;0.8090169943749469;0.15643446504023453;-0.95105651629515442;0.70710678118654602;0.30901699437494862;-0.98768834059513833;-0.30901699437494673;0.95105651629515364 ...(+7561 chars)])"  SampleTime=1.953125e-06  TableDataTypeStr=fixdt(1,18,16)
  crp_out_delay{,1..23} (24 alike) : Delay  DelayLength=1  InitialCondition=0  SampleTime=1.953125e-06
  crp_temp_shared : Subsystem
  crp_temp_shared1 : Subsystem
  crp_temp_shared2 : Subsystem
  crp_temp_shared3 : Subsystem
  crp_temp_shared4 : Subsystem
  crp_temp_shared5 : Subsystem
  crp_temp_shared6 : Subsystem
  crp_temp_shared7 : Subsystem
  crp_temp_shared8 : Subsystem
  crp_temp_shared9 : Subsystem
  delayMatch{,1,3..4,6..7,9..10,12..15,17..18,21..24,27..28,31..34,37..40,43..44,48..49,52..53,56..57,60..61,64..65} (40 alike) : Delay  DelayLength=1  InitialCondition=0  SampleTime=1.953125e-06
  delayMatch{66..103} (38 alike) : Delay  DelayLength=1  InitialCondition=0  SampleTime=0.000125
  delayMatch{2,5,8,11,16,19} (6 alike) : Delay  DelayLength=65  InitialCondition=0  SampleTime=1.953125e-06
  delayMatch{20,25..26,29..30,35..36} (7 alike) : Delay  DelayLength=25  InitialCondition=0  SampleTime=1.953125e-06
  delayMatch{41..42,46..47,50..51,54..55,58..59,62..63} (12 alike) : Delay  DelayLength=64  InitialCondition=0  SampleTime=1.953125e-06
  delayMatch45 : Delay  DelayLength=9  InitialCondition=0  SampleTime=1.953125e-06
  in0_repeat : RateTransition  Integrity=off  Deterministic=off  OutPortSampleTimeOpt=Multiple of input port sample time  OutPortSampleTimeMultiple=1/64
  in10_repeat : RateTransition  Integrity=off  Deterministic=off  OutPortSampleTimeOpt=Multiple of input port sample time  OutPortSampleTimeMultiple=1/64
  in11_repeat : RateTransition  Integrity=off  Deterministic=off  OutPortSampleTimeOpt=Multiple of input port sample time  OutPortSampleTimeMultiple=1/64
  in12_repeat : RateTransition  Integrity=off  Deterministic=off  OutPortSampleTimeOpt=Multiple of input port sample time  OutPortSampleTimeMultiple=1/64
  in13_repeat : RateTransition  Integrity=off  Deterministic=off  OutPortSampleTimeOpt=Multiple of input port sample time  OutPortSampleTimeMultiple=1/64
  in14_repeat : RateTransition  Integrity=off  Deterministic=off  OutPortSampleTimeOpt=Multiple of input port sample time  OutPortSampleTimeMultiple=1/64
  in15_repeat : RateTransition  Integrity=off  Deterministic=off  OutPortSampleTimeOpt=Multiple of input port sample time  OutPortSampleTimeMultiple=1/64
  in16_repeat : RateTransition  Integrity=off  Deterministic=off  OutPortSampleTimeOpt=Multiple of input port sample time  OutPortSampleTimeMultiple=1/64
  in18_repeat : RateTransition  Integrity=off  Deterministic=off  OutPortSampleTimeOpt=Multiple of input port sample time  OutPortSampleTimeMultiple=1/64
  in19_repeat : RateTransition  Integrity=off  Deterministic=off  OutPortSampleTimeOpt=Multiple of input port sample time  OutPortSampleTimeMultiple=1/64
  in20_repeat : RateTransition  Integrity=off  Deterministic=off  OutPortSampleTimeOpt=Multiple of input port sample time  OutPortSampleTimeMultiple=1/64
  in21_repeat : RateTransition  Integrity=off  Deterministic=off  OutPortSampleTimeOpt=Multiple of input port sample time  OutPortSampleTimeMultiple=1/64
  in22_repeat : RateTransition  Integrity=off  Deterministic=off  OutPortSampleTimeOpt=Multiple of input port sample time  OutPortSampleTimeMultiple=1/64
  in23_repeat : RateTransition  Integrity=off  Deterministic=off  OutPortSampleTimeOpt=Multiple of input port sample time  OutPortSampleTimeMultiple=1/64
  in24_repeat : RateTransition  Integrity=off  Deterministic=off  OutPortSampleTimeOpt=Multiple of input port sample time  OutPortSampleTimeMultiple=1/64
  in25_repeat : RateTransition  Integrity=off  Deterministic=off  OutPortSampleTimeOpt=Multiple of input port sample time  OutPortSampleTimeMultiple=1/64
  in27_repeat : RateTransition  Integrity=off  Deterministic=off  OutPortSampleTimeOpt=Multiple of input port sample time  OutPortSampleTimeMultiple=1/64
  in28_repeat : RateTransition  Integrity=off  Deterministic=off  OutPortSampleTimeOpt=Multiple of input port sample time  OutPortSampleTimeMultiple=1/64
  in29_repeat : RateTransition  Integrity=off  Deterministic=off  OutPortSampleTimeOpt=Multiple of input port sample time  OutPortSampleTimeMultiple=1/64
  in2_repeat : RateTransition  Integrity=off  Deterministic=off  OutPortSampleTimeOpt=Multiple of input port sample time  OutPortSampleTimeMultiple=1/64
  in30_repeat : RateTransition  Integrity=off  Deterministic=off  OutPortSampleTimeOpt=Multiple of input port sample time  OutPortSampleTimeMultiple=1/64
  in31_repeat : RateTransition  Integrity=off  Deterministic=off  OutPortSampleTimeOpt=Multiple of input port sample time  OutPortSampleTimeMultiple=1/64
  in32_repeat : RateTransition  Integrity=off  Deterministic=off  OutPortSampleTimeOpt=Multiple of input port sample time  OutPortSampleTimeMultiple=1/64
  in33_repeat : RateTransition  Integrity=off  Deterministic=off  OutPortSampleTimeOpt=Multiple of input port sample time  OutPortSampleTimeMultiple=1/64
  in34_repeat : RateTransition  Integrity=off  Deterministic=off  OutPortSampleTimeOpt=Multiple of input port sample time  OutPortSampleTimeMultiple=1/64
  in36_repeat : RateTransition  Integrity=off  Deterministic=off  OutPortSampleTimeOpt=Multiple of input port sample time  OutPortSampleTimeMultiple=1/64
  in37_repeat : RateTransition  Integrity=off  Deterministic=off  OutPortSampleTimeOpt=Multiple of input port sample time  OutPortSampleTimeMultiple=1/64
  in38_repeat : RateTransition  Integrity=off  Deterministic=off  OutPortSampleTimeOpt=Multiple of input port sample time  OutPortSampleTimeMultiple=1/64
  in39_repeat : RateTransition  Integrity=off  Deterministic=off  OutPortSampleTimeOpt=Multiple of input port sample time  OutPortSampleTimeMultiple=1/64
  in3_repeat : RateTransition  Integrity=off  Deterministic=off  OutPortSampleTimeOpt=Multiple of input port sample time  OutPortSampleTimeMultiple=1/64
  in40_repeat : RateTransition  Integrity=off  Deterministic=off  OutPortSampleTimeOpt=Multiple of input port sample time  OutPortSampleTimeMultiple=1/64
  in41_repeat : RateTransition  Integrity=off  Deterministic=off  OutPortSampleTimeOpt=Multiple of input port sample time  OutPortSampleTimeMultiple=1/64
  in42_repeat : RateTransition  Integrity=off  Deterministic=off  OutPortSampleTimeOpt=Multiple of input port sample time  OutPortSampleTimeMultiple=1/64
  in43_repeat : RateTransition  Integrity=off  Deterministic=off  OutPortSampleTimeOpt=Multiple of input port sample time  OutPortSampleTimeMultiple=1/64
  in44_repeat : RateTransition  Integrity=off  Deterministic=off  OutPortSampleTimeOpt=Multiple of input port sample time  OutPortSampleTimeMultiple=1/64
  in45_repeat : RateTransition  Integrity=off  Deterministic=off  OutPortSampleTimeOpt=Multiple of input port sample time  OutPortSampleTimeMultiple=1/64
  in46_repeat : RateTransition  Integrity=off  Deterministic=off  OutPortSampleTimeOpt=Multiple of input port sample time  OutPortSampleTimeMultiple=1/64
  in47_repeat : RateTransition  Integrity=off  Deterministic=off  OutPortSampleTimeOpt=Multiple of input port sample time  OutPortSampleTimeMultiple=1/64
  in49_repeat : RateTransition  Integrity=off  Deterministic=off  OutPortSampleTimeOpt=Multiple of input port sample time  OutPortSampleTimeMultiple=1/64
  in4_repeat : RateTransition  Integrity=off  Deterministic=off  OutPortSampleTimeOpt=Multiple of input port sample time  OutPortSampleTimeMultiple=1/64
  in50_repeat : RateTransition  Integrity=off  Deterministic=off  OutPortSampleTimeOpt=Multiple of input port sample time  OutPortSampleTimeMultiple=1/64
  in51_repeat : RateTransition  Integrity=off  Deterministic=off  OutPortSampleTimeOpt=Multiple of input port sample time  OutPortSampleTimeMultiple=1/64
  in52_repeat : RateTransition  Integrity=off  Deterministic=off  OutPortSampleTimeOpt=Multiple of input port sample time  OutPortSampleTimeMultiple=1/64
  in53_repeat : RateTransition  Integrity=off  Deterministic=off  OutPortSampleTimeOpt=Multiple of input port sample time  OutPortSampleTimeMultiple=1/64
  in54_repeat : RateTransition  Integrity=off  Deterministic=off  OutPortSampleTimeOpt=Multiple of input port sample time  OutPortSampleTimeMultiple=1/64
  in55_repeat : RateTransition  Integrity=off  Deterministic=off  OutPortSampleTimeOpt=Multiple of input port sample time  OutPortSampleTimeMultiple=1/64
  in56_repeat : RateTransition  Integrity=off  Deterministic=off  OutPortSampleTimeOpt=Multiple of input port sample time  OutPortSampleTimeMultiple=1/64
  in57_repeat : RateTransition  Integrity=off  Deterministic=off  OutPortSampleTimeOpt=Multiple of input port sample time  OutPortSampleTimeMultiple=1/64
  in5_repeat : RateTransition  Integrity=off  Deterministic=off  OutPortSampleTimeOpt=Multiple of input port sample time  OutPortSampleTimeMultiple=1/64
  in6_repeat : RateTransition  Integrity=off  Deterministic=off  OutPortSampleTimeOpt=Multiple of input port sample time  OutPortSampleTimeMultiple=1/64
  in7_repeat : RateTransition  Integrity=off  Deterministic=off  OutPortSampleTimeOpt=Multiple of input port sample time  OutPortSampleTimeMultiple=1/64
  in8_repeat : RateTransition  Integrity=off  Deterministic=off  OutPortSampleTimeOpt=Multiple of input port sample time  OutPortSampleTimeMultiple=1/64
  in9_repeat : RateTransition  Integrity=off  Deterministic=off  OutPortSampleTimeOpt=Multiple of input port sample time  OutPortSampleTimeMultiple=1/64
  na1_1_out_dtc{,1..7} (8 alike) : DataTypeConversion  OutDataTypeStr=fixdt(1, 40, 30)  SampleTime=1.953125e-06  RndMeth=Floor
  na1_2_out_dtc{,1..7} (8 alike) : DataTypeConversion  OutDataTypeStr=fixdt(1, 40, 30)  SampleTime=1.953125e-06  RndMeth=Floor
  na2_1_out_dtc{,1..7} (8 alike) : DataTypeConversion  OutDataTypeStr=fixdt(1, 40, 30)  SampleTime=1.953125e-06  RndMeth=Floor
  na2_2_out_dtc{,1..7} (8 alike) : DataTypeConversion  OutDataTypeStr=fixdt(1, 40, 30)  SampleTime=1.953125e-06  RndMeth=Floor
  out0_bypass{,1..37} (38 alike) : UnitDelay  SampleTime=0.000125
  reset_in{,1..5} (6 alike) : Switch  Criteria=u2 ~= 0  OutDataTypeStr=fixdt(1, 32, 30)  SampleTime=1.953125e-06  SaturateOnIntegerOverflow=off  InputSameDT=off
  reset_out{,1..5} (6 alike) : Switch  Criteria=u2 ~= 0  OutDataTypeStr=fixdt(1, 32, 30)  SampleTime=1.953125e-06  SaturateOnIntegerOverflow=off  InputSameDT=off
  sinLUT{,1..3} (4 alike) : LookupNDDirect  Table="reshape([0;0;0;0;0;0;0;0;0;0;0;0;0;0;0;0;0.3090169943749474;0.45399049973954675;0.58778525229247314;0.70710678118654746;0.80901699437494745;0.89100652418836779;0.95105651629515353;0.98768834059513777;1;0.98768834059513777;0.95105651629515364;0.8910065241883679;0.80901699437494745;0.70710678118654757;0.58778525229247325;0.45399049973954686;0.58778525229247314;0.80901699437494745;0.95105651629515353;1;0.95105651629515364;0.80901699437494745;0.58778525229247325;0.30901699437494751;1.2246467991473532e-16;-0.30901699437494728;-0.58778525229247303;-0.80901699437494734;-0.95105651629515353;-1;-0.95105651629515364;-0.80901699437494756;0.80901699437494745;0.98768834059513777;0.95105651629515364;0.70710678118654757;0.30901699437494751;-0.15643446504023031;-0.58778525229247303;-0.89100652418836779;-1;-0.89100652418836801;-0.58778525229247336;-0.15643446504023198;0.30901699437494634;0.70710678118654668;0.95105651629515353;0.98768834059513788;0.95105651629515353;0.95105651629515364;0.58778525229247325;1.2246467991473532e-16;-0.58778525229247303;-0.95105651629515353;-0.95105651629515364;-0.58778525229247336;-2.4492935982947064e-16;0.58778525229247292;0.95105651629515353;0.95105651629515364;0.58778525229247336;3.6739403974420594e-16;-0.5877852522924728;-0.95105651629515342;1;0.70710678118654757;-3.2162452993532732e-16;-0.70710678118654713;-1;-0.70710678118654768;6.4324905987065464e-16;0.70710678118654668;1;0.70710678118654713;3.6739403974420594e-16;-0.70710678118654657;-1;-0.70710678118654724;1.2864981197413093e-15;0.70710678118654657;0.95105651629515364;0.30901699437494751;-0.58778525229247303;-1;-0.58778525229247336;0.30901699437494634;0.95105651629515353;0.80901699437494756;3.6739403974420594e-16;-0.80901699437494723;-0.95105651629515375;-0.30901699437494956;0.58778525229247125;1;0.58778525229247358;-0.30901699437494512;0.80901699437494723;-0.15643446504023073;-0.95105651629515375;-0.70710678118654768;0.30901699437494717;0.98768834059513755;0.58778525229247192;-0.45399049973954725;-1;-0.45399049973954642;0.58778525229247269;0.98768834059513799;0.30901699437494967;-0.70710678118654768;-0.95105651629515264;-0.15643446504023248;0.58778525229247325;-0.58778525229247303;-0.95105651629515364;-2.4492935982947064e-16;0.95105651629515353;0.58778525229247336;-0.5877852522924728;-0.95105651629515375;-4.8985871965894128e-16;0.95105651629515342;0.58778525229247358;-0.58778525229247258;-0.95105651629515375;-7.3478807948841188e-16;0.95105651629515331;0.5877852522924738;0.30901699437494751;-0.89100652418836779;-0.58778525229247336;0.70710678118654668;0.80901699437494756;-0.45399049973954564;-0.95105651629515375;0.15643446504022951;1;0.15643446504023059;-0.95105651629515342;-0.4539904997395498;0.8090169943749459;0.70710678118654879;-0.58778525229247247;-0.8910065241883679;-3.2162452993532732e-16;-1;6.4324905987065464e-16;1;3.6739403974420594e-16;-1;1.2864981197413093e-15;1;2.388680238973927e-15;-1;-7.3478807948841188e-16;1;8.5725275940314722e-16;-1;2.5729962394826186e-15;1;-0.30901699437494728;-0.89100652418836834;0.58778525229247292;0.70710678118654835;-0.80901699437494612;-0.45399049973954803;0.95105651629515342;0.15643446504023059;-1;0.15643446504023101;0.95105651629515497;-0.45399049973954519;-0.80901699437494901;0.70710678118654746;0.58778525229247403;-0.89100652418836535;-0.58778525229247303;-0.58778525229247336;0.95105651629515353;3.6739403974420594e-16;-0.95105651629515375;0.58778525229247125;0.58778525229247358;-0.95105651629515342;-7.3478807948841188e-16;0.95105651629515386;-0.58778525229247247;-0.5877852522924768;0.9510565162951522;4.6548957980331188e-15;-0.95105651629515398;0.58778525229246925;-0.80901699437494734;-0.15643446504023112;0.95105651629515364;-0.70710678118654657;-0.3090169943749479;0.98768834059513799;-0.58778525229247258;-0.45399049973954664;1;-0.45399049973954841;-0.58778525229247391;0.9876883405951371;-0.30901699437494468;-0.70710678118654902;0.9510565162951532;-0.1564344650402269;-0.95105651629515375;0.30901699437494717 ...(+7874 chars)])"  SampleTime=1.953125e-06  TableDataTypeStr=fixdt(1,18,16)
  stateControl{,1..37} (38 alike) : Constant  OutDataTypeStr=boolean  SampleTime=0.000125
  P_theta : Outport  OutDataTypeStr=fixdt(0, 40, 34)  PortDimensions=1  SampleTime=1.953125e-06
  wires:
  Product_out_dtc4/1 -> Add8/1
  cosLUT/1 -> PipelineRegister4/1
  delayMatch4/1 -> Add3/2
  b0_1_out_dtc/1 -> S0_1/1
  D1_16/1 -> S1_1_out1bypassMux6/1
  out0_bypass14/1 -> S2_2_out1bypassMux2/3
  crp_temp_shared4/3(out2) -> na1_1_out_dtc6/1
  cosLUT2/1 -> PipelineRegister7/1
  in15_repeat/1 -> delayMatch12/1
  Product1_out_dtc12/1 -> crp_temp_shared2/1(in0)
  delayMatch49/1 -> Delay_Switch/3
  delayMatch17/1 -> Minus4/2
  delayMatch19/1 -> reset_in5/2
  PipelineRegister10/1 -> crp_temp_shared1/2(in1)
  S1_2_stage34/1 -> crp_out_delay15/1
  S1_2_stage24/1 -> S1_2_stage34/1
  in49_repeat/1 -> delayMatch38/1
  Product1_out_dtc/1 -> Add13/2
  cosLUT3/1 -> PipelineRegister9/1
  D2_1_absorbed2/1 -> in29_repeat/1
  in12_repeat/1 -> reset_out/3
  out0_bypass13/1 -> S1_2_out1bypassMux1/3
  delayMatch6/1 -> Minus1/2
  sinLUT/1 -> PipelineRegister3/1
  Delay_lowered_absorbed1/1 -> in12_repeat/1
  Delay_lowered/1 -> Delay_toDelbypassMux/1
  sinLUT3/1 -> PipelineRegister10/1
  S2_22/1 -> D2_22/1
  S1_1_out1bypassMux5/1 -> out0_bypass28/1, D1_1_absorbed5/1
  crp_temp_shared5/9(out8) -> b0_2_out_dtc5/1
  out0_bypass11/1 -> S2_1_out1bypassMux1/3
  Minus2/1 -> Gain3/1
  Product3_out_dtc/1 -> Add11/2
  delayMatch21/1 -> S1_1_stage31/2
  sinLUT2/1 -> PipelineRegister8/1
  delayMatch65/1 -> Delay_Switch4/3
  Delay2_bypass/1 -> in5_repeat/1
  Product_out_dtc13/1 -> Add21/1
  b0_1_out_dtc6/1 -> delayMatch45/1
  out0_bypass24/1 -> S1_1_out1bypassMux4/3
  Minus1/1 -> Gain2/1
  in9_repeat/1 -> delayMatch44/1, bypass_out3/1
  delayMatch55/1 -> reset_out2/2
  S1_2_stage32/1 -> D1_22/1
  Add4/1 -> reset_in2/3
  S2_1_out1bypassMux4/1 -> out0_bypass23/1, D2_1_absorbed4/1
  IdxConv15/1 -> Direct Lookup Table (n-D)/2
  stateControl14/1 -> delayMatch80/1
  Direct Lookup Table (n-D)3/1 -> PipelineRegister/1
  stateControl13/1 -> delayMatch79/1
  IdxConv12/1 -> cosLUT2/2
  crp_temp_shared/9(out8) -> Product_out_dtc/1
  b0_1_out_dtc3/1 -> S0_13/1
  sinLUT1/1 -> PipelineRegister5/1
  S2_12/1 -> crp_out_delay6/1
  cosLUT1/1 -> PipelineRegister6/1
  D1_24/1 -> S1_2_out1bypassMux4/1
  S1_2_stage3/1 -> crp_out_delay3/1
  stateControl/1 -> delayMatch66/1
  in21_repeat/1 -> bypass_out5/1, delayMatch61/1
  reset_in1/1 -> Delay_lowered1/1
  Gain2/1 -> Add4/1
  stateControl22/1 -> delayMatch88/1
  Add11/1 -> Add1_stage3/2
  na2_2_out_dtc5/1 -> S2_25/2
  S1_2_out1bypassMux3/1 -> out0_bypass21/1, D1_2_absorbed3/1
  delayMatch8/1 -> reset_in2/2
  na2_1_out_dtc4/1 -> S2_14/2
  D1_1_absorbed7/1 -> in52_repeat/1
  delayMatch37/1 -> S1_1_stage36/2
  Direct Lookup Table (n-D)1/1 -> PipelineRegister1/1
  in18_repeat/1 -> IdxConv13/1, IdxConv12/1, IdxConv11/1, IdxConv1/1, IdxConv33/1, IdxConv32/1, IdxConv34/1, IdxConv31/1
  delayMatch22/1 -> S1_2_stage31/2
  stateControl28/1 -> delayMatch94/1
  delayMatch1/1 -> Add2/2
  Q_17/1 -> crp_temp_shared5/2(in1)
  crp_temp_shared8/11(out10) -> Product1_out_dtc10/1
  delayMatch40/1 -> S1_2_stage37/2
  Constant1/1 -> Compare/2
  crp_temp_shared4/11(out10) -> b1_2_out_dtc3/1
  b0_1_out_dtc4/1 -> S0_14/1
  D2_2/1 -> S2_2_out1bypassMux/1
  delayMatch25/1 -> S2_13/1
  S2_27/1 -> D2_27/1
  b1_1_out_dtc4/1 -> delayMatch30/1
  delayMatch39/1 -> S1_1_stage37/2
  delayMatch90/1 -> S1_1_out1bypassMux4/2
  S1_2_stage27/1 -> S1_2_stage37/1
  S1_1_stage23/1 -> S1_1_stage33/1
  b1_1_out_dtc6/1 -> delayMatch36/1
  Product1_out_dtc1/1 -> Add/2
  crp_temp_shared8/13(out12) -> na2_2_out_dtc2/1
  delayMatch77/1 -> S2_1_out1bypassMux1/2
  crp_temp_shared/12(out11) -> Product2_out_dtc1/1
  delayMatch36/1 -> S1_1_stage26/1
  delayMatch38/1 -> S1_2_stage36/2
  S0_1/1 -> Q_1/1
  crp_temp_shared3/1(out0) -> b0_1_out_dtc1/1
  IdxConv9/1 -> cosLUT2/1
  delayMatch87/1 -> S1_2_out1bypassMux3/2
  S1_2_out1bypassMux2/1 -> D1_2_absorbed2/1, out0_bypass17/1
  delayMatch56/1 -> Delay_Switch2/2
  delayMatch33/1 -> S1_1_stage35/2
  na2_2_out_dtc7/1 -> S2_27/2
  crp_temp_shared1/2(out1) -> Product_out_dtc9/1
  delayMatch94/1 -> S1_1_out1bypassMux5/2
  S1_1_out1bypassMux6/1 -> out0_bypass32/1, D1_1_absorbed6/1
  delayMatch35/1 -> S2_16/1
  b2_2_out_dtc7/1 -> S2_27/1
  IdxConv23/1 -> sinLUT2/1
  crp_temp_shared4/8(out7) -> na1_1_out_dtc4/1
  reset_out2/1 -> delayMatch10/1, delayMatch9/1, Delay_Switch2/1
  b0_2_out_dtc1/1 -> S0_21/1
  crp_out_delay18/1 -> D2_26/1
  stateControl18/1 -> delayMatch84/1
  crp_temp_shared/3(out2) -> Product1_out_dtc2/1
  Compare/1 -> bypass_out2/2, bypass_out1/2, bypass_out4/2, delayMatch60/1, delayMatch56/1, delayMatch64/1, bypass_out5/2, delayMatch52/1, delayMatch43/1, bypass_out/2, bypass_out3/2, delayMatch48/1
  S2_2/1 -> D2_2/1
  crp_temp_shared5/4(out3) -> b0_2_out_dtc7/1
  delayMatch34/1 -> S1_2_stage35/2
  na2_1_out_dtc1/1 -> S2_11/2
  crp_temp_shared2/5(out4) -> Gain1_out_dtc/1
  Delay_toDelbypassMux/1 -> out0_bypass/1, Delay_lowered_absorbed/1
  out0_bypass36/1 -> S1_1_out1bypassMux7/3
  b0_2_out_dtc6/1 -> S0_26/1
  stateControl34/1 -> delayMatch100/1
  crp_temp_shared9/2(out1) -> Product_out_dtc6/1
  delayMatch79/1 -> S1_2_out1bypassMux1/2
  delayMatch5/1 -> reset_in1/2
  out0_bypass30/1 -> S2_2_out1bypassMux6/3
  in11_repeat/1 -> delayMatch63/1, delayMatch51/1, delayMatch42/1, delayMatch8/1, delayMatch5/1, delayMatch2/1, delayMatch19/1, delayMatch55/1, delayMatch16/1, delayMatch59/1, delayMatch47/1, delayMatch11/1
  b2_2_out_dtc2/1 -> S2_22/1
  S0_16/1 -> Q_16/1
  delayMatch32/1 -> S1_2_stage34/2
  D1_1/1 -> S1_1_out1bypassMux/1
  Q_2/1 -> crp_temp_shared9/1(in0), crp_temp_shared8/5(in4)
  crp_temp_shared3/15(out14) -> b2_2_out_dtc6/1
  delayMatch31/1 -> S1_1_stage34/2
  Product1_out_dtc13/1 -> Add21/2
  Gain4/1 -> Add6/1
  b2_1_out_dtc2/1 -> S2_12/1
  stateControl37/1 -> delayMatch103/1
  S1_2_stage23/1 -> S1_2_stage33/1
  Product1_out_dtc8/1 -> Add9/2
  crp_temp_shared5/16(out15) -> na2_1_out_dtc2/1
  delayMatch29/1 -> S2_14/1
  delayMatch81/1 -> S2_1_out1bypassMux2/2
  Delay1_lowered/1 -> Delay1_lowered_absorbed/1
  na1_2_out_dtc4/1 -> S1_2_stage24/2
  Q_15/1 -> crp_temp_shared5/3(in2)
  PipelineRegister7/1 -> crp_temp_shared1/7(in6)
  delayMatch66/1 -> Delay_toDelbypassMux/2
  crp_temp_shared/7(out6) -> Product1_out_dtc/1
  D1_2_absorbed2/1 -> in32_repeat/1
  delayMatch51/1 -> reset_out1/2
  D2_2_absorbed6/1 -> in49_repeat/1
  D2_17/1 -> S2_1_out1bypassMux7/1
  crp_out_delay20/1 -> D1_16/1
  crp_temp_shared2/7(out6) -> b2_1_out_dtc6/1
  crp_temp_shared1/7(out6) -> Product_out_dtc2/1
  delayMatch28/1 -> S1_2_stage33/2
  S1_2_stage26/1 -> S1_2_stage36/1
  S1_1_stage22/1 -> S1_1_stage32/1
  bypass_out5/1 -> Delay_bypass1/1, crp_temp_shared/1(in0)
  delayMatch27/1 -> S1_1_stage33/2
  b2_1_out_dtc4/1 -> delayMatch29/1
  out0_bypass21/1 -> S1_2_out1bypassMux3/3
  delayMatch26/1 -> S1_1_stage23/1
  Subtract3/1 -> Minus5/1
  D2_2_absorbed7/1 -> in53_repeat/1
  stateControl29/1 -> delayMatch95/1
  na2_1_out_dtc6/1 -> S2_16/2
  Q_12/1 -> crp_temp_shared5/4(in3), crp_temp_shared6/1(in0)
  F0 Index/1 -> IdxConv14/1, IdxConv4/1, IdxConv2/1, IdxConv6/1, IdxConv24/1, IdxConv9/1, IdxConv22/1, IdxConv10/1, IdxConv/1, IdxConv23/1, IdxConv8/1, IdxConv21/1
  crp_out_delay6/1 -> D2_12/1
  Gain14/1 -> crp_temp_shared2/7(in6)
  delayMatch46/1 -> reset_out/1
  delayMatch83/1 -> S1_2_out1bypassMux2/2
  b1_2_out_dtc6/1 -> S1_2_stage26/1
  delayMatch24/1 -> S1_2_stage32/2
  delayMatch23/1 -> S1_1_stage32/2
  IdxConv8/1 -> cosLUT1/1
  crp_out_delay2/1 -> D1_1/1
  in0_repeat/1 -> bypass_out4/1, delayMatch65/1
  Delay_toDelbypassMux5/1 -> out0_bypass9/1, Delay_lowered_absorbed6/1
  delayMatch9/1 -> Minus2/2
  crp_temp_shared8/8(out7) -> na2_2_out_dtc5/1
  D1_1_absorbed3/1 -> in34_repeat/1
  crp_temp_shared5/3(out2) -> b2_2_out_dtc7/1
  in23_repeat/1 -> reset_out4/3
  crp_out_delay14/1 -> D1_14/1
  crp_temp_shared8/4(out3) -> Product1_out_dtc4/1
  crp_temp_shared8/1(out0) -> Product_out_dtc4/1
  D1_15/1 -> S1_1_out1bypassMux5/1
  delayMatch18/1 -> Add7/2
  delayMatch42/1 -> reset_out5/2
  Add13/1 -> Add_stage2/1
  out0_bypass35/1 -> S2_1_out1bypassMux7/3
  S2_21/1 -> D2_21/1
  delayMatch64/1 -> Delay_Switch4/2
  na1_2_out_dtc2/1 -> S1_2_stage22/2
  reset_out4/1 -> Delay_Switch4/1, delayMatch18/1, delayMatch17/1
  Delay_lowered_absorbed5/1 -> in21_repeat/1
  out0_bypass18/1 -> S2_2_out1bypassMux3/3
  S0_14/1 -> Q_14/1
  na1_1_out_dtc2/1 -> S1_1_stage22/2
  delayMatch16/1 -> reset_in4/2
  delayMatch70/1 -> S2_2_out1bypassMux/2
  crp_temp_shared1/5(out4) -> Product_out_dtc5/1
  delayMatch11/1 -> reset_in3/2
  out0_bypass25/1 -> S1_2_out1bypassMux4/3
  b1_1_out_dtc2/1 -> S1_1_stage22/1
  delayMatch15/1 -> Add6/2
  PipelineRegister6/1 -> crp_temp_shared1/8(in7)
  crp_temp_shared5/13(out12) -> b2_2_out_dtc2/1
  Mic3/1 -> crp_temp_shared1/6(in5)
  crp_temp_shared6/10(out9) -> na2_2_out_dtc4/1
  b1_1_out_dtc3/1 -> delayMatch26/1
  crp_temp_shared2/6(out5) -> Gain_out_dtc/1
  delayMatch92/1 -> S2_2_out1bypassMux5/2
  in56_repeat/1 -> bypass_out4/3
  delayMatch14/1 -> Minus3/2
  b0_2_out_dtc3/1 -> S0_23/1
  stateControl4/1 -> delayMatch70/1
  crp_temp_shared2/9(out8) -> b1_1_out_dtc6/1
  delayMatch63/1 -> reset_out4/2
  IdxConv32/1 -> sinLUT1/2
  Q_26/1 -> crp_temp_shared8/6(in5), crp_temp_shared6/3(in2)
  crp_temp_shared4/7(out6) -> na2_1_out_dtc4/1
  Gain/1 -> Add2/1
  S2_2_out1bypassMux6/1 -> D2_2_absorbed6/1, out0_bypass30/1
  Delay2_lowered_absorbed/1 -> in4_repeat/1
  D1_2/1 -> S1_2_out1bypassMux/1
  IdxConv10/1 -> cosLUT3/1
  stateControl27/1 -> delayMatch93/1
  IdxConv/1 -> cosLUT/1
  delayMatch60/1 -> Delay_Switch3/2
  in2_repeat/1 -> bypass_out/1, delayMatch57/1
  crp_temp_shared5/8(out7) -> b2_2_out_dtc5/1
  Q_21/1 -> crp_temp_shared8/1(in0)
  Delay_lowered_absorbed4/1 -> in22_repeat/1
  IdxConv13/1 -> cosLUT3/2
  b2_1_out_dtc3/1 -> delayMatch25/1
  delayMatch72/1 -> S1_1_out1bypassMux/2
  delayMatch13/1 -> S1_2_stage3/2
  D2_21/1 -> S2_2_out1bypassMux1/1
  in54_repeat/1 -> S0_27/2
  delayMatch12/1 -> S1_1_stage3/2
  sch_ctr_63/1 -> crp_temp_shared9/3(enb_counter), crp_temp_shared8/8(enb_counter), crp_temp_shared4/5(enb_counter), crp_temp_shared2/11(enb_counter), crp_temp_shared3/7(enb_counter), crp_temp_shared/11(enb_counter), crp_temp_shared5/5(enb_counter), crp_temp_shared7/3(enb_counter), crp_temp_shared1/13(enb_counter), crp_temp_shared6/8(enb_counter)
  S1_2_out1bypassMux5/1 -> D1_2_absorbed5/1, out0_bypass29/1
  in52_repeat/1 -> S0_17/2
  out0_bypass15/1 -> S2_1_out1bypassMux2/3
  delayMatch10/1 -> Add5/2
  S1_1_stage3/1 -> crp_out_delay2/1
  delayMatch3/1 -> Minus/2
  Product1_out_dtc5/1 -> crp_temp_shared2/3(in2)
  reset_out3/1 -> delayMatch15/1, Delay_Switch3/1, delayMatch14/1
  stateControl25/1 -> delayMatch91/1
  D2_2_absorbed/1 -> in19_repeat/1
  delayMatch59/1 -> reset_out3/2
  Product_out_dtc12/1 -> Add13/1
  crp_temp_shared2/2(out1) -> Gain_out_dtc3/1
  delayMatch103/1 -> S1_2_out1bypassMux7/2
  Gain5/1 -> Add7/1
  delayMatch7/1 -> Add4/2
  S1_1_out1bypassMux2/1 -> out0_bypass16/1, D1_1_absorbed2/1
  S1_2_stage33/1 -> crp_out_delay11/1
  delayMatch52/1 -> Delay_Switch1/2
  crp_temp_shared6/2(out1) -> b2_2_out_dtc/1
  bypass_out3/1 -> crp_temp_shared/2(in1), Delay5_bypass1/1
  crp_temp_shared2/14(out13) -> b0_1_out_dtc3/1
  in20_repeat/1 -> S0_2/2
  reset_out/1 -> delayMatch4/1, Delay_Switch/1, delayMatch3/1
  delayMatch2/1 -> reset_in/2
  crp_temp_shared5/11(out10) -> na2_1_out_dtc5/1
  delayMatch/1 -> Minus5/2
  Delay3_bypass1/1 -> Delay3_bypass/1
  S0_23/1 -> Q_23/1
  Add12/1 -> Add1_stage2/1
  stateControl23/1 -> delayMatch89/1
  out0_bypass5/1 -> S2_1_out1bypassMux/3
  S0_21/1 -> Q_21/1
  Q_14/1 -> crp_temp_shared4/2(in1)
  na1_2_out_dtc7/1 -> S1_2_stage27/2
  D2_25/1 -> S2_2_out1bypassMux5/1
  in5_repeat/1 -> bypass_out1/3
  PipelineRegister9/1 -> crp_temp_shared1/3(in2)
  Product_out_dtc3/1 -> Subtract1/1
  crp_temp_shared4/10(out9) -> b0_2_out_dtc3/1
  out0_bypass2/1 -> Delay_toDelbypassMux2/3
  in27_repeat/1 -> delayMatch22/1
  delayMatch48/1 -> Delay_Switch/2
  D2_16/1 -> S2_1_out1bypassMux6/1
  S1_1_out1bypassMux4/1 -> out0_bypass24/1, D1_1_absorbed4/1
  Product_out_dtc9/1 -> Gain14/1
  delayMatch47/1 -> reset_out/2
  b1_2_out_dtc4/1 -> S1_2_stage24/1
  crp_out_delay10/1 -> D1_13/1
  IdxConv6/1 -> Direct Lookup Table (n-D)3/1
  Delay4_lowered/1 -> Delay4_lowered_absorbed/1
  PipelineRegister/1 -> Switch/1, crp_temp_shared2/6(in5)
  Product3_out_dtc1/1 -> Add12/2
  delayMatch100/1 -> S2_2_out1bypassMux7/2
  crp_temp_shared1/8(out7) -> Product1_out_dtc3/1
  crp_out_delay21/1 -> D1_26/1
  b2_1_out_dtc7/1 -> S2_17/1
  crp_temp_shared8/2(out1) -> na2_2_out_dtc1/1
  stateControl6/1 -> delayMatch72/1
  Add_stage2/1 -> Add_stage3/1
  delayMatch99/1 -> S1_2_out1bypassMux6/2
  S2_2_out1bypassMux5/1 -> out0_bypass26/1, D2_2_absorbed5/1
  Mic1/1 -> crp_temp_shared1/4(in3)
  PipelineRegister5/1 -> crp_temp_shared1/10(in9)
  b2_1_out_dtc6/1 -> delayMatch35/1
  crp_out_delay11/1 -> D1_23/1
  stateControl32/1 -> delayMatch98/1
  b2_1_out_dtc5/1 -> S2_15/1
  out0_bypass19/1 -> S2_1_out1bypassMux3/3
  S2_16/1 -> crp_out_delay19/1
  S2_2_out1bypassMux1/1 -> D2_2_absorbed1/1, out0_bypass10/1
  A Counter/1 -> in6_repeat/1
  b2_2_out_dtc5/1 -> S2_25/1
  bypass_out4/1 -> crp_temp_shared/4(in3), Delay1_bypass1/1
  b2_2_out_dtc4/1 -> S2_24/1
  IdxConv2/1 -> Direct Lookup Table (n-D)1/1
  b0_2_out_dtc/1 -> S0_2/1
  Initial_Val/1 -> reset_in/1, delayMatch41/1
  S0_2/1 -> Q_2/1
  stateControl20/1 -> delayMatch86/1
  b1_2_out_dtc3/1 -> S1_2_stage23/1
  crp_out_delay12/1 -> D2_24/1
  Minus5/1 -> Gain/1
  stateControl16/1 -> delayMatch82/1
  crp_temp_shared8/14(out13) -> na1_2_out_dtc2/1
  Delay1_bypass1/1 -> Delay1_bypass/1
  Product1_out_dtc11/1 -> Add10/2
  Delay_lowered1/1 -> Delay_toDelbypassMux1/1
  b2_2_out_dtc3/1 -> S2_23/1
  S2_11/1 -> crp_out_delay4/1
  crp_temp_shared2/15(out14) -> b1_1_out_dtc3/1
  S2_24/1 -> crp_out_delay12/1
  Abs/1 -> IdxConv15/1, IdxConv7/1, IdxConv3/1, IdxConv5/1
  na2_2_out_dtc6/1 -> S2_26/2
  Gain3/1 -> Add5/1
  Add8/1 -> Minus3/1
  stateControl24/1 -> delayMatch90/1
  in39_repeat/1 -> S0_14/2
  na2_2_out_dtc1/1 -> S2_21/2
  in42_repeat/1 -> delayMatch33/1
  Product_out_dtc1/1 -> Add1/1
  Add2/1 -> reset_in/3
  in50_repeat/1 -> S0_26/2
  Gain_out_dtc/1 -> Switch/3
  b1_1_out_dtc1/1 -> S1_1_stage21/1
  out0_bypass/1 -> Delay_toDelbypassMux/3
  b2_1_out_dtc1/1 -> delayMatch20/1
  crp_out_delay/1 -> Delay_lowered3/1
  S1_1_out1bypassMux3/1 -> out0_bypass20/1, D1_1_absorbed3/1
  b2_2_out_dtc1/1 -> S2_21/1
  in25_repeat/1 -> S0_11/2
  Delay_toDelbypassMux2/1 -> out0_bypass2/1, Delay_lowered_absorbed2/1
  PipelineRegister2/1 -> crp_temp_shared/7(in6)
  b1_2_out_dtc5/1 -> S1_2_stage25/1
  IdxConv4/1 -> Direct Lookup Table (n-D)2/1
  S2_14/1 -> crp_out_delay13/1
  Product_out_dtc2/1 -> Gain11/1
  Add6/1 -> reset_in4/3
  crp_temp_shared/11(out10) -> Product2_out_dtc/1
  b2_1_out_dtc/1 -> S2_1/1
  b2_2_out_dtc/1 -> S2_2/1
  Product1_out_dtc7/1 -> Subtract2/2
  crp_out_delay9/1 -> D2_13/1
  b0_2_out_dtc5/1 -> S0_25/1
  Delay_lowered_absorbed3/1 -> in14_repeat/1
  Minus3/1 -> Gain4/1
  delayMatch76/1 -> S2_2_out1bypassMux1/2
  na1_1_out_dtc6/1 -> S1_1_stage26/2
  na1_2_out_dtc/1 -> S1_2_stage2/2
  Product_out_dtc11/1 -> Subtract3/1
  IdxConv33/1 -> sinLUT2/2
  S2_26/1 -> crp_out_delay18/1
  D1_1_absorbed2/1 -> in30_repeat/1
  crp_temp_shared4/4(out3) -> b2_2_out_dtc4/1
  Gain13/1 -> crp_temp_shared2/8(in7)
  na2_2_out_dtc4/1 -> S2_24/2
  crp_temp_shared5/12(out11) -> na1_1_out_dtc5/1
  Add/1 -> Add_stage2/2
  stateControl30/1 -> delayMatch96/1
  Add7/1 -> reset_in5/3
  Product_out_dtc/1 -> Add/1
  D2_11/1 -> S2_1_out1bypassMux1/1
  na2_1_out_dtc3/1 -> S2_13/2
  Gain12/1 -> crp_temp_shared2/9(in8)
  out0_bypass29/1 -> S1_2_out1bypassMux5/3
  Minus/1 -> Gain1/1
  S0_11/1 -> Q_11/1
  delayMatch71/1 -> S2_1_out1bypassMux/2
  Product2_out_dtc1/1 -> Add11/1
  crp_temp_shared6/4(out3) -> b1_2_out_dtc/1
  in44_repeat/1 -> delayMatch34/1
  Add14/1 -> Add1_stage2/2
  out0_bypass4/1 -> S2_2_out1bypassMux/3
  Product2_out_dtc/1 -> Add14/1
  Product2_out_dtc2/1 -> Add12/1
  delayMatch57/1 -> Delay_Switch2/3
  D1_26/1 -> S1_2_out1bypassMux6/1
  delayMatch50/1 -> reset_out1/1
  crp_temp_shared7/1(out0) -> Product1_out_dtc13/1
  D1_1_absorbed/1 -> in16_repeat/1
  crp_temp_shared/6(out5) -> Product3_out_dtc2/1
  crp_temp_shared7/2(out1) -> Product_out_dtc13/1
  Add1_stage3/1 -> crp_temp_shared7/1(in0)
  in32_repeat/1 -> S0_22/2
  crp_temp_shared5/10(out9) -> b1_2_out_dtc5/1
  crp_temp_shared/2(out1) -> Product_out_dtc12/1
  crp_temp_shared/1(out0) -> Product2_out_dtc2/1
  crp_temp_shared/8(out7) -> Product3_out_dtc1/1
  S2_15/1 -> crp_out_delay16/1
  S1_1_stage21/1 -> S1_1_stage31/1
  D2_1_absorbed6/1 -> in46_repeat/1
  crp_temp_shared4/2(out1) -> na2_1_out_dtc6/1
  crp_temp_shared6/7(out6) -> na2_2_out_dtc6/1
  S2_2_out1bypassMux7/1 -> out0_bypass34/1, D2_2_absorbed7/1
  stateControl7/1 -> delayMatch73/1
  out0_bypass1/1 -> Delay_toDelbypassMux1/3
  D1_17/1 -> S1_1_out1bypassMux7/1
  reset_in3/1 -> crp_out_delay/1
  S1_1_stage32/1 -> crp_out_delay7/1
  delayMatch68/1 -> Delay_toDelbypassMux2/2
  crp_temp_shared/10(out9) -> Product_out_dtc1/1
  crp_temp_shared3/3(out2) -> b2_1_out_dtc7/1
  S1_2_out1bypassMux4/1 -> out0_bypass25/1, D1_2_absorbed4/1
  crp_temp_shared5/7(out6) -> na1_1_out_dtc7/1
  Delay_Switch2/1 -> Delay3_lowered/1
  crp_temp_shared8/7(out6) -> Product1_out_dtc11/1
  crp_temp_shared4/1(out0) -> b1_2_out_dtc6/1
  Delay_toDelbypassMux3/1 -> out0_bypass3/1, Delay_lowered_absorbed3/1
  delayMatch91/1 -> S1_2_out1bypassMux4/2
  Delay_lowered_absorbed2/1 -> in13_repeat/1
  na2_1_out_dtc2/1 -> S2_12/2
  crp_out_delay22/1 -> D2_17/1
  out0_bypass12/1 -> S1_1_out1bypassMux1/3
  crp_temp_shared1/4(out3) -> Product_out_dtc7/1
  na1_2_out_dtc1/1 -> S1_2_stage21/2
  crp_temp_shared4/14(out13) -> b2_2_out_dtc1/1
  delayMatch43/1 -> Delay_Switch5/2
  out0_bypass3/1 -> Delay_toDelbypassMux3/3
  crp_temp_shared3/6(out5) -> b2_1_out_dtc5/1
  out0_bypass33/1 -> S1_2_out1bypassMux6/3
  delayMatch98/1 -> S1_1_out1bypassMux6/2
  crp_temp_shared4/9(out8) -> b2_2_out_dtc3/1
  crp_temp_shared8/10(out9) -> Product1_out_dtc8/1
  Delay3_lowered/1 -> Delay3_lowered_absorbed/1
  S0_13/1 -> Q_13/1
  S0_27/1 -> Q_27/1
  Product_out_dtc7/1 -> Gain13/1
  crp_temp_shared6/12(out11) -> Product_out_dtc8/1
  S1_1_out1bypassMux7/1 -> out0_bypass36/1, D1_1_absorbed7/1
  crp_temp_shared4/5(out4) -> b0_2_out_dtc4/1
  Delay_toDelbypassMux4/1 -> out0_bypass8/1, Delay_lowered_absorbed4/1
  delayMatch62/1 -> reset_out4/1
  Delay2_bypass1/1 -> Delay2_bypass/1
  crp_temp_shared2/10(out9) -> b2_1_out_dtc4/1
  in29_repeat/1 -> delayMatch23/1
  IdxConv14/1 -> Direct Lookup Table (n-D)/1
  Minus4/1 -> Gain5/1
  S0_25/1 -> Q_25/1
  S1_1_stage31/1 -> crp_out_delay5/1
  in38_repeat/1 -> delayMatch31/1
  crp_temp_shared3/12(out11) -> b2_1_out_dtc/1
  crp_temp_shared3/11(out10) -> b1_1_out_dtc2/1
  out0_bypass37/1 -> S1_2_out1bypassMux7/3
  S0_15/1 -> Q_15/1
  Product1_out_dtc2/1 -> Add1/2
  crp_temp_shared2/13(out12) -> b2_1_out_dtc3/1
  S1_2_stage2/1 -> S1_2_stage3/1
  D2_2_absorbed5/1 -> in44_repeat/1
  delayMatch88/1 -> S2_2_out1bypassMux4/2
  S0_26/1 -> Q_26/1
  S0_12/1 -> Q_12/1
  na1_1_out_dtc3/1 -> S1_1_stage23/2
  crp_temp_shared6/15(out14) -> na1_2_out_dtc3/1
  crp_temp_shared8/12(out11) -> Product1_out_dtc6/1
  na1_1_out_dtc/1 -> S1_1_stage2/2
  crp_temp_shared3/10(out9) -> b0_1_out_dtc2/1
  Delay4_bypass1/1 -> Delay4_bypass/1
  IdxConv7/1 -> Direct Lookup Table (n-D)3/2
  crp_temp_shared3/9(out8) -> b2_1_out_dtc2/1
  out0_bypass16/1 -> S1_1_out1bypassMux2/3
  S0_24/1 -> Q_24/1
  crp_temp_shared6/1(out0) -> na1_1_out_dtc2/1
  stateControl11/1 -> delayMatch77/1
  Product1_out_dtc10/1 -> Subtract3/2
  crp_temp_shared8/15(out14) -> Product_out_dtc3/1
  delayMatch75/1 -> Delay_toDelbypassMux5/2
  Add1_stage2/1 -> Add1_stage3/1
  out0_bypass9/1 -> Delay_toDelbypassMux5/3
  crp_temp_shared2/16(out15) -> b2_1_out_dtc1/1
  out0_bypass31/1 -> S2_1_out1bypassMux6/3
  crp_temp_shared4/13(out12) -> na1_1_out_dtc3/1
  D2_1_absorbed5/1 -> in42_repeat/1
  crp_temp_shared3/2(out1) -> b1_1_out_dtc1/1
  S1_1_stage27/1 -> S1_1_stage37/1
  Q_11/1 -> crp_temp_shared5/1(in0), crp_temp_shared4/4(in3)
  S1_2_stage22/1 -> S1_2_stage32/1
  na2_1_out_dtc5/1 -> S2_15/2
  na2_2_out_dtc/1 -> S2_2/2
  crp_temp_shared2/8(out7) -> b0_1_out_dtc6/1
  stateControl10/1 -> delayMatch76/1
  out0_bypass34/1 -> S2_2_out1bypassMux7/3
  Product_out_dtc8/1 -> Add9/1
  crp_temp_shared/4(out3) -> Product3_out_dtc/1
  crp_temp_shared/5(out4) -> Product1_out_dtc1/1
  S1_1_stage26/1 -> S1_1_stage36/1
  S1_2_stage25/1 -> S1_2_stage35/1
  S1_1_stage25/1 -> S1_1_stage35/1
  D2_13/1 -> S2_1_out1bypassMux3/1
  S1_1_stage24/1 -> S1_1_stage34/1
  IdxConv24/1 -> sinLUT3/1
  in24_repeat/1 -> delayMatch21/1
  Product_out_dtc5/1 -> Gain12/1
  out0_bypass7/1 -> S1_2_out1bypassMux/3
  reset_out1/1 -> delayMatch7/1, delayMatch6/1, Delay_Switch1/1
  S1_2_stage21/1 -> S1_2_stage31/1
  S1_1_stage2/1 -> S1_1_stage3/1
  Delay1_lowered_absorbed/1 -> in0_repeat/1
  Product3_out_dtc2/1 -> Add14/2
  delayMatch61/1 -> Delay_Switch3/3
  delayMatch44/1 -> Delay_Switch5/3
  na2_1_out_dtc7/1 -> S2_17/2
  D1_14/1 -> S1_1_out1bypassMux4/1
  delayMatch53/1 -> Delay_Switch1/3
  out0_bypass17/1 -> S1_2_out1bypassMux2/3
  delayMatch86/1 -> S1_1_out1bypassMux3/2
  b2_2_out_dtc6/1 -> S2_26/1
  crp_out_delay7/1 -> D1_12/1
  IdxConv5/1 -> Direct Lookup Table (n-D)2/2
  na1_2_out_dtc5/1 -> S1_2_stage25/2
  reset_in/1 -> Delay_lowered/1
  out0_bypass22/1 -> S2_2_out1bypassMux4/3
  Add_stage3/1 -> crp_temp_shared7/2(in1)
  S2_23/1 -> crp_out_delay8/1
  in30_repeat/1 -> S0_12/2
  stateControl12/1 -> delayMatch78/1
  out0_bypass32/1 -> S1_1_out1bypassMux6/3
  Add10/1 -> Minus/1
  D2_22/1 -> S2_2_out1bypassMux2/1
  out0_bypass27/1 -> S2_1_out1bypassMux5/3
  D2_14/1 -> S2_1_out1bypassMux4/1
  S2_17/1 -> crp_out_delay22/1
  Delay4_bypass/1 -> in8_repeat/1
  S1_1_stage36/1 -> crp_out_delay20/1
  Product1_out_dtc6/1 -> Add8/2
  Q_22/1 -> crp_temp_shared8/7(in6)
  IdxConv34/1 -> sinLUT3/2
  delayMatch84/1 -> S2_2_out1bypassMux3/2
  crp_temp_shared2/11(out10) -> b0_1_out_dtc4/1
  S0_17/1 -> Q_17/1
  S1_1_stage37/1 -> crp_out_delay23/1
  na1_1_out_dtc7/1 -> S1_1_stage27/2
  Gain1/1 -> Add3/1
  S1_2_stage36/1 -> crp_out_delay21/1
  Subtract1/1 -> Minus4/1
  Add5/1 -> reset_in3/3
  na1_2_out_dtc6/1 -> S1_2_stage26/2
  S1_2_stage35/1 -> D1_25/1
  Product1_out_dtc4/1 -> Subtract1/2
  Product1_out_dtc9/1 -> crp_temp_shared2/2(in1)
  crp_temp_shared2/1(out0) -> Gain_out_dtc4/1
  PipelineRegister8/1 -> crp_temp_shared1/5(in4)
  delayMatch93/1 -> S2_1_out1bypassMux5/2
  b0_1_out_dtc5/1 -> S0_15/1
  delayMatch58/1 -> reset_out3/1
  S1_1_stage35/1 -> crp_out_delay17/1
  na1_1_out_dtc5/1 -> S1_1_stage25/2
  Add9/1 -> Minus1/1
  Q_24/1 -> crp_temp_shared6/5(in4)
  Direct Lookup Table (n-D)/1 -> PipelineRegister11/1
  D1_2_absorbed3/1 -> in37_repeat/1
  b0_2_out_dtc4/1 -> S0_24/1
  na1_1_out_dtc4/1 -> S1_1_stage24/2
  Delay5_bypass/1 -> in10_repeat/1
  D2_23/1 -> S2_2_out1bypassMux3/1
  Subtract/1 -> Abs/1
  D1_2_absorbed1/1 -> in28_repeat/1
  na2_2_out_dtc2/1 -> S2_22/2
  S1_1_stage34/1 -> crp_out_delay14/1
  crp_temp_shared6/6(out5) -> na1_1_out_dtc/1
  Subtract2/1 -> Minus2/1
  Product_out_dtc6/1 -> Subtract2/1
  na2_2_out_dtc3/1 -> S2_23/2
  delayMatch41/1 -> reset_out5/1
  Q_13/1 -> crp_temp_shared4/3(in2)
  in55_repeat/1 -> reset_out5/3
  Q_16/1 -> crp_temp_shared4/1(in0), crp_temp_shared3/6(in5)
  na1_2_out_dtc3/1 -> S1_2_stage23/2
  S2_13/1 -> crp_out_delay9/1
  Product_out_dtc10/1 -> Add10/1
  in57_repeat/1 -> bypass_out5/3
  IdxConv11/1 -> cosLUT1/2
  delayMatch89/1 -> S2_1_out1bypassMux4/2
  crp_temp_shared3/8(out7) -> b1_1_out_dtc5/1
  S1_1_stage33/1 -> crp_out_delay10/1
  out0_bypass20/1 -> S1_1_out1bypassMux3/3
  na1_1_out_dtc1/1 -> S1_1_stage21/2
  IdxConv22/1 -> sinLUT1/1
  crp_temp_shared8/16(out15) -> na2_2_out_dtc/1
  Gain1_out_dtc/1 -> Switch1/3
  PipelineRegister4/1 -> crp_temp_shared1/11(in10)
  Delay_lowered_absorbed/1 -> in55_repeat/1
  IdxConv1/1 -> cosLUT/2
  in41_repeat/1 -> S0_24/2
  na2_1_out_dtc/1 -> S2_1/2
  S2_1/1 -> crp_out_delay1/1
  PipelineRegister3/1 -> crp_temp_shared1/12(in11)
  crp_temp_shared3/14(out13) -> b1_1_out_dtc/1
  out0_bypass6/1 -> S1_1_out1bypassMux/3
  Delay_Switch1/1 -> Delay2_lowered/1
  D1_1_absorbed6/1 -> in47_repeat/1
  IdxConv31/1 -> sinLUT/2
  IdxConv21/1 -> sinLUT/1
  Gain11/1 -> crp_temp_shared3/1(in0), crp_temp_shared2/10(in9)
  stateControl35/1 -> delayMatch101/1
  delayMatch54/1 -> reset_out2/1
  crp_temp_shared6/16(out15) -> Product_out_dtc11/1
  S2_1_out1bypassMux7/1 -> out0_bypass35/1, D2_1_absorbed7/1
  in7_repeat/1 -> bypass_out2/1, delayMatch49/1
  Constant/1 -> Relational Operator/2, Subtract/2
  IdxConv3/1 -> Direct Lookup Table (n-D)1/2
  out0_bypass10/1 -> S2_2_out1bypassMux1/3
  S1_1_out1bypassMux1/1 -> out0_bypass12/1, D1_1_absorbed1/1
  delayMatch85/1 -> S2_1_out1bypassMux3/2
  out0_bypass28/1 -> S1_1_out1bypassMux5/3
  out0_bypass26/1 -> S2_2_out1bypassMux5/3
  out0_bypass23/1 -> S2_1_out1bypassMux4/3
  D1_2_absorbed4/1 -> in41_repeat/1
  Delay2_lowered/1 -> Delay2_lowered_absorbed/1
  out0_bypass8/1 -> Delay_toDelbypassMux4/3
  D1_21/1 -> S1_2_out1bypassMux1/1
  S1_2_out1bypassMux/1 -> out0_bypass7/1, D1_2_absorbed/1
  delayMatch101/1 -> S2_1_out1bypassMux7/2
  D2_2_absorbed1/1 -> in27_repeat/1
  delayMatch102/1 -> S1_1_out1bypassMux7/2
  delayMatch97/1 -> S2_1_out1bypassMux6/2
  delayMatch96/1 -> S2_2_out1bypassMux6/2
  S1_2_out1bypassMux1/1 -> out0_bypass13/1, D1_2_absorbed1/1
  crp_temp_shared6/11(out10) -> na1_2_out_dtc4/1
  delayMatch95/1 -> S1_2_out1bypassMux5/2
  IQ Counter/1 -> in18_repeat/1
  delayMatch82/1 -> S1_1_out1bypassMux2/2
  crp_temp_shared3/4(out3) -> b0_1_out_dtc7/1
  delayMatch80/1 -> S2_2_out1bypassMux2/2
  bypass_out2/1 -> crp_temp_shared/8(in7), Delay4_bypass1/1
  delayMatch78/1 -> S1_1_out1bypassMux1/2
  delayMatch74/1 -> Delay_toDelbypassMux4/2
  delayMatch73/1 -> S1_2_out1bypassMux/2
  delayMatch69/1 -> Delay_toDelbypassMux3/2
  delayMatch67/1 -> Delay_toDelbypassMux1/2
  Delay_toDelbypassMux1/1 -> out0_bypass1/1, Delay_lowered_absorbed1/1
  D1_27/1 -> S1_2_out1bypassMux7/1
  stateControl1/1 -> delayMatch67/1
  stateControl8/1 -> delayMatch74/1
  in13_repeat/1 -> reset_out1/3
  D2_27/1 -> S2_2_out1bypassMux7/1
  D1_2_absorbed6/1 -> in50_repeat/1
  crp_out_delay1/1 -> D2_1/1
  D2_26/1 -> S2_2_out1bypassMux6/1
  D1_25/1 -> S1_2_out1bypassMux5/1
  D2_15/1 -> S2_1_out1bypassMux5/1
  D2_24/1 -> S2_2_out1bypassMux4/1
  D1_23/1 -> S1_2_out1bypassMux3/1
  S1_2_stage37/1 -> D1_27/1
  S2_1_out1bypassMux2/1 -> out0_bypass15/1, D2_1_absorbed2/1
  D1_13/1 -> S1_1_out1bypassMux3/1
  D1_22/1 -> S1_2_out1bypassMux2/1
  D1_12/1 -> S1_1_out1bypassMux2/1
  D2_12/1 -> S2_1_out1bypassMux2/1
  stateControl36/1 -> delayMatch102/1
  in47_repeat/1 -> S0_16/2
  Q_23/1 -> crp_temp_shared9/2(in1), crp_temp_shared8/2(in1), crp_temp_shared6/4(in3)
  D1_11/1 -> S1_1_out1bypassMux1/1
  Delay_lowered6/1 -> Delay_toDelbypassMux5/1
  Delay_lowered4/1 -> Delay_toDelbypassMux4/1
  Delay4_lowered_absorbed/1 -> in7_repeat/1
  D2_1/1 -> S2_1_out1bypassMux/1
  Delay_lowered3/1 -> Delay_toDelbypassMux3/1
  Delay_Switch/1 -> Delay4_lowered/1
  Delay_lowered2/1 -> Delay_toDelbypassMux2/1
  crp_out_delay19/1 -> D2_16/1
  stateControl33/1 -> delayMatch99/1
  stateControl31/1 -> delayMatch97/1
  Delay5_lowered_absorbed/1 -> in9_repeat/1
  stateControl26/1 -> delayMatch92/1
  S2_25/1 -> D2_25/1
  stateControl21/1 -> delayMatch87/1
  stateControl19/1 -> delayMatch85/1
  Mic2/1 -> crp_temp_shared1/9(in8)
  stateControl17/1 -> delayMatch83/1
  stateControl15/1 -> delayMatch81/1
  S1_2_stage31/1 -> D1_21/1
  Direct Lookup Table (n-D)2/1 -> PipelineRegister2/1
  stateControl9/1 -> delayMatch75/1
  reset_in5/1 -> Delay_lowered6/1
  reset_in4/1 -> Delay_lowered4/1
  S0_22/1 -> Q_22/1
  stateControl5/1 -> delayMatch71/1
  stateControl3/1 -> delayMatch69/1
  D2_1_absorbed1/1 -> in24_repeat/1
  stateControl2/1 -> delayMatch68/1
  reset_in2/1 -> Delay_lowered2/1
  crp_out_delay23/1 -> D1_17/1
  Q_1/1 -> crp_temp_shared6/2(in1)
  Initial_Val2/1 -> reset_in2/1, delayMatch50/1
  crp_out_delay17/1 -> D1_15/1
  bypass_out1/1 -> crp_temp_shared/6(in5), Delay2_bypass1/1
  crp_temp_shared5/5(out4) -> b1_2_out_dtc7/1
  crp_out_delay16/1 -> D2_15/1
  b1_2_out_dtc7/1 -> S1_2_stage27/1
  crp_out_delay15/1 -> D1_24/1
  crp_out_delay13/1 -> D2_14/1
  crp_out_delay8/1 -> D2_23/1
  crp_out_delay5/1 -> D1_11/1
  crp_out_delay4/1 -> D2_11/1
  crp_temp_shared3/16(out15) -> b0_2_out_dtc6/1
  Delay_Switch4/1 -> Delay1_lowered/1
  Delay_Switch3/1 -> Delay_lowered5/1
  crp_out_delay3/1 -> D1_2/1
  Delay_Switch5/1 -> Delay5_lowered/1
  in53_repeat/1 -> delayMatch40/1
  in51_repeat/1 -> delayMatch39/1
  in46_repeat/1 -> delayMatch37/1
  in45_repeat/1 -> S0_25/2
  in43_repeat/1 -> S0_15/2
  in40_repeat/1 -> delayMatch32/1
  in37_repeat/1 -> S0_23/2
  S2_1_out1bypassMux/1 -> out0_bypass5/1, D2_1_absorbed/1
  in36_repeat/1 -> delayMatch28/1
  in34_repeat/1 -> S0_13/2
  in33_repeat/1 -> delayMatch27/1
  in31_repeat/1 -> delayMatch24/1
  in8_repeat/1 -> bypass_out2/3
  in28_repeat/1 -> S0_21/2
  in19_repeat/1 -> delayMatch13/1
  in16_repeat/1 -> S0_1/2
  in10_repeat/1 -> bypass_out3/3
  in3_repeat/1 -> bypass_out/3
  Delay_lowered5/1 -> Delay_lowered_absorbed5/1
  Delay5_lowered/1 -> Delay5_lowered_absorbed/1
  Delay5_bypass1/1 -> Delay5_bypass/1
  Delay_bypass1/1 -> Delay_bypass/1
  D1_2_absorbed7/1 -> in54_repeat/1
  D2_1_absorbed7/1 -> in51_repeat/1
  D1_2_absorbed5/1 -> in45_repeat/1
  D1_1_absorbed5/1 -> in43_repeat/1
  D1_1_absorbed4/1 -> in39_repeat/1
  D2_1_absorbed4/1 -> in38_repeat/1
  D2_2_absorbed4/1 -> in40_repeat/1
  crp_temp_shared1/6(out5) -> Product1_out_dtc5/1
  D2_1_absorbed3/1 -> in33_repeat/1
  D2_2_absorbed3/1 -> in36_repeat/1
  Initial_Val5/1 -> reset_in5/1, delayMatch62/1
  D2_2_absorbed2/1 -> in31_repeat/1
  D1_1_absorbed1/1 -> in25_repeat/1
  Delay_lowered_absorbed6/1 -> in23_repeat/1
  D1_2_absorbed/1 -> in20_repeat/1
  Delay3_bypass/1 -> in3_repeat/1
  D2_1_absorbed/1 -> in15_repeat/1
  Mic4/1 -> crp_temp_shared1/1(in0)
  Initial_Val1/1 -> reset_in1/1, delayMatch46/1
  RESET/1 -> in11_repeat/1
  Add21/1 -> P_theta/1
  Initial_Val4/1 -> reset_in4/1, delayMatch58/1
  Initial_Val3/1 -> reset_in3/1, delayMatch54/1
  reset_out5/1 -> delayMatch1/1, delayMatch/1, Delay_Switch5/1
  Relational Operator/1 -> Switch1/2, Switch/2
  PipelineRegister1/1 -> Switch1/1, crp_temp_shared2/5(in4)
  Q_27/1 -> crp_temp_shared8/4(in3), crp_temp_shared6/7(in6)
  Q_25/1 -> crp_temp_shared8/3(in2), crp_temp_shared6/6(in5)
  S1_2_out1bypassMux7/1 -> out0_bypass37/1, D1_2_absorbed7/1
  S1_2_out1bypassMux6/1 -> out0_bypass33/1, D1_2_absorbed6/1
  crp_temp_shared6/3(out2) -> b0_2_out_dtc/1
  S2_1_out1bypassMux6/1 -> out0_bypass31/1, D2_1_absorbed6/1
  S2_1_out1bypassMux5/1 -> out0_bypass27/1, D2_1_absorbed5/1
  S2_2_out1bypassMux4/1 -> out0_bypass22/1, D2_2_absorbed4/1
  S2_1_out1bypassMux3/1 -> out0_bypass19/1, D2_1_absorbed3/1
  S2_2_out1bypassMux3/1 -> out0_bypass18/1, D2_2_absorbed3/1
  S2_2_out1bypassMux2/1 -> out0_bypass14/1, D2_2_absorbed2/1
  S2_1_out1bypassMux1/1 -> out0_bypass11/1, D2_1_absorbed1/1
  S1_1_out1bypassMux/1 -> out0_bypass6/1, D1_1_absorbed/1
  Add1/1 -> Add_stage3/2
  S2_2_out1bypassMux/1 -> out0_bypass4/1, D2_2_absorbed/1
  bypass_out/1 -> Delay3_bypass1/1, crp_temp_shared/3(in2)
  in6_repeat/1 -> Compare/1, Relational Operator/1, Subtract/1
  in4_repeat/1 -> delayMatch53/1, bypass_out1/1
  crp_temp_shared1/3(out2) -> Product1_out_dtc9/1
  delayMatch45/1 -> S0_16/1
  PipelineRegister11/1 -> crp_temp_shared/5(in4)
  crp_temp_shared1/1(out0) -> Product1_out_dtc12/1
  Gain_out_dtc1/1 -> crp_temp_shared3/5(in4)
  crp_temp_shared2/12(out11) -> b1_1_out_dtc4/1
  Product1_out_dtc3/1 -> crp_temp_shared2/4(in3)
  Gain_out_dtc3/1 -> crp_temp_shared3/3(in2)
  crp_temp_shared2/3(out2) -> Gain_out_dtc2/1
  Switch/1 -> crp_temp_shared/10(in9)
  crp_temp_shared2/4(out3) -> Gain_out_dtc1/1
  Switch1/1 -> crp_temp_shared/9(in8)
  delayMatch20/1 -> S2_11/1
  Gain_out_dtc2/1 -> crp_temp_shared3/4(in3)
  crp_temp_shared3/7(out6) -> b0_1_out_dtc5/1
  Gain_out_dtc4/1 -> crp_temp_shared3/2(in1)
  delayMatch30/1 -> S1_1_stage24/1
  crp_temp_shared3/5(out4) -> b1_1_out_dtc7/1
  crp_temp_shared4/6(out5) -> b1_2_out_dtc4/1
  crp_temp_shared3/13(out12) -> b0_1_out_dtc/1
  b1_1_out_dtc/1 -> S1_1_stage2/1
  b1_1_out_dtc7/1 -> S1_1_stage27/1
  b0_2_out_dtc7/1 -> S0_27/1
  b0_1_out_dtc1/1 -> S0_11/1
  b1_1_out_dtc5/1 -> S1_1_stage25/1
  b0_1_out_dtc7/1 -> S0_17/1
  b0_1_out_dtc2/1 -> S0_12/1
  b1_2_out_dtc1/1 -> S1_2_stage21/1
  crp_temp_shared5/15(out14) -> b1_2_out_dtc2/1
  crp_temp_shared4/15(out14) -> b0_2_out_dtc1/1
  crp_temp_shared4/16(out15) -> b1_2_out_dtc1/1
  b1_2_out_dtc/1 -> S1_2_stage2/1
  crp_temp_shared5/14(out13) -> b0_2_out_dtc2/1
  b0_2_out_dtc2/1 -> S0_22/1
  b1_2_out_dtc2/1 -> S1_2_stage22/1
  crp_temp_shared6/9(out8) -> Product_out_dtc10/1
  crp_temp_shared6/13(out12) -> Product1_out_dtc7/1
  crp_temp_shared6/5(out4) -> na2_1_out_dtc/1
  Add3/1 -> reset_in1/3
  Delay1_bypass/1 -> in56_repeat/1
  crp_temp_shared4/12(out11) -> na2_1_out_dtc3/1
  Delay3_lowered_absorbed/1 -> in2_repeat/1
  crp_temp_shared6/8(out7) -> na1_2_out_dtc6/1
  Delay_bypass/1 -> in57_repeat/1
  crp_temp_shared5/2(out1) -> na1_1_out_dtc1/1
  crp_temp_shared5/1(out0) -> na2_1_out_dtc1/1
  crp_temp_shared5/6(out5) -> na2_1_out_dtc7/1
  crp_temp_shared6/14(out13) -> na2_2_out_dtc3/1
  crp_temp_shared8/3(out2) -> na1_2_out_dtc1/1
  crp_temp_shared8/5(out4) -> na2_2_out_dtc7/1
  crp_temp_shared8/6(out5) -> na1_2_out_dtc7/1
  crp_temp_shared8/9(out8) -> na1_2_out_dtc5/1
  crp_temp_shared9/1(out0) -> na1_2_out_dtc/1
  in14_repeat/1 -> reset_out2/3
  in22_repeat/1 -> reset_out3/3
